simulink model "NBMS_App_Harness1"  (R2026b)
settings: Solver=FixedStepDiscrete  StopTime=25  FixedStep=0.1
undefined symbols (not defined in the file): Active_DisChrg_E, BMS_BattSoCDerate_E, BMS_BattTempDerate_E, BMS_DCDCMosfet_STS_E, BMS_HVMosfet_STS_E, BMS_MODE_E, BMS_NM_Msg_E, BMS_PMosfet_STS_E, Charger_Mode_E, Charger_Mode_Req_E, CV_Mode_Timer_E, OBC_E, VDU_MACHINE_STS_E
(part 4 of 4)

== stateflow chart NBMS_App_Harness1/Test Assessment ==
  state ChargeWhenIgOn
    state step_1
      if t < 0.2
      Expected_BMSMODE = BMS_MODE_E.BMS_SLEEP;
      elseif t >= 0.2 && t < 0.4
      Expected_BMSMODE = BMS_MODE_E.BMS_STANDBY;
      else
      Expected_BMSMODE = BMS_MODE_E.BMS_CHARGE;
      end
      if t < 1.1
      Expected_PrechgMosfet = BMS_PMosfet_STS_E.PDISCONNECTED;
      elseif t >= 1.1 && t < 2.7
      Expected_PrechgMosfet = BMS_PMosfet_STS_E.PCONNECTED;
      else
      Expected_PrechgMosfet = BMS_PMosfet_STS_E.PDISCONNECTED;
      end
      if t < 1.7
      Expected_HVMosfet = BMS_HVMosfet_STS_E.HV_DISCONNECTED;
      elseif t >= 1.7 && t < 2.7
      Expected_HVMosfet = BMS_HVMosfet_STS_E.HV_CONNECT_PENDING;
      else
      Expected_HVMosfet = BMS_HVMosfet_STS_E.HV_CONNECTED;
      end
      if t < 2.2
      Expected_DCDCMosfet = BMS_DCDCMosfet_STS_E.DCDC_DISCONNECTED;
      else
      Expected_DCDCMosfet = BMS_DCDCMosfet_STS_E.DCDC_CONNECTED;
      end
      Expected_ASC_Prep_Flag = false;
      Expected_Chrgr_Prep_Flag = false;
      Expected_PrechgVoltFlt = false;
      verify(AppOut_BMSMODE == Expected_BMSMODE);
      verify(AppOut_PrechgMosfet == Expected_PrechgMosfet);
      verify(AppOut_HVMosfet == Expected_HVMosfet);
      verify(AppOut_DCDCMosfet == Expected_DCDCMosfet);
      verify(AppOut_ASC_Prep_Flag == Expected_ASC_Prep_Flag);
      verify(AppOut_Chrgr_Prep_Flag == Expected_Chrgr_Prep_Flag);
      verify(AppOut_PrechgVoltFlt == Expected_PrechgVoltFlt);
    (default) -> ChargeWhenIgOn.step_1
  state DischgWhenIgOn
    state step_1
      if t < 0.2
      Expected_BMSMODE  = BMS_MODE_E.BMS_SLEEP;
      elseif t >= 0.2 && t < 0.4
      Expected_BMSMODE  = BMS_MODE_E.BMS_STANDBY;
      else
      Expected_BMSMODE  = BMS_MODE_E.BMS_DISCHARGE;
      end
      if t < 1.1
      Expected_PrechgMosfet = BMS_PMosfet_STS_E.PDISCONNECTED;
      elseif t >= 1.1 && t < 2.8
      Expected_PrechgMosfet = BMS_PMosfet_STS_E.PCONNECTED;
      else
      Expected_PrechgMosfet = BMS_PMosfet_STS_E.PDISCONNECTED;
      end
      if t < 1.8
      Expected_HVMosfet = BMS_HVMosfet_STS_E.HV_DISCONNECTED;
      elseif t >= 1.8 && t < 2.8
      Expected_HVMosfet = BMS_HVMosfet_STS_E.HV_CONNECT_PENDING;
      else
      Expected_HVMosfet = BMS_HVMosfet_STS_E.HV_CONNECTED;
      end
      if t < 2.3
      Expected_DCDCMosfet = BMS_DCDCMosfet_STS_E.DCDC_DISCONNECTED;
      else
      Expected_DCDCMosfet = BMS_DCDCMosfet_STS_E.DCDC_CONNECTED;
      end
      Expected_ASC_Prep_Flag = false;
      Expected_Chrgr_Prep_Flag = false;
      Expected_PrechgVoltFlt = false;
      verify(AppOut_BMSMODE == Expected_BMSMODE );
      verify(AppOut_PrechgMosfet == Expected_PrechgMosfet);
      verify(AppOut_HVMosfet == Expected_HVMosfet);
      verify(AppOut_DCDCMosfet == Expected_DCDCMosfet);
      verify(AppOut_ASC_Prep_Flag == Expected_ASC_Prep_Flag);
      verify(AppOut_Chrgr_Prep_Flag == Expected_Chrgr_Prep_Flag);
      verify(AppOut_PrechgVoltFlt == Expected_PrechgVoltFlt);
    (default) -> DischgWhenIgOn.step_1
  state ChargeWhenIgOff
    state step_1
      if t < 0.2
      Expected_BMSMODE  = BMS_MODE_E.BMS_SLEEP;
      elseif t >= 0.2 && t < 0.3
      Expected_BMSMODE  = BMS_MODE_E.BMS_STANDBY;
      else
      Expected_BMSMODE  = BMS_MODE_E.BMS_CHARGE;
      end
      if t < 0.9
      Expected_PrechgMosfet = BMS_PMosfet_STS_E.PDISCONNECTED;
      elseif t >= 0.9 && t < 2.4
      Expected_PrechgMosfet = BMS_PMosfet_STS_E.PCONNECTED;
      else
      Expected_PrechgMosfet = BMS_PMosfet_STS_E.PDISCONNECTED;
      end
      if t < 1.9
      Expected_HVMosfet = BMS_HVMosfet_STS_E.HV_DISCONNECTED;
      elseif t >= 1.9 && t < 2.4
      Expected_HVMosfet = BMS_HVMosfet_STS_E.HV_CONNECT_PENDING;
      else
      Expected_HVMosfet = BMS_HVMosfet_STS_E.HV_CONNECTED;
      end
      Expected_DCDCMosfet = BMS_DCDCMosfet_STS_E.DCDC_DISCONNECTED;
      Expected_ASC_Prep_Flag = false;
      Expected_Chrgr_Prep_Flag = false;
      Expected_PrechgVoltFlt = false;
      verify(AppOut_BMSMODE == Expected_BMSMODE );
      verify(AppOut_PrechgMosfet == Expected_PrechgMosfet);
      verify(AppOut_HVMosfet == Expected_HVMosfet);
      verify(AppOut_DCDCMosfet == Expected_DCDCMosfet);
      verify(AppOut_ASC_Prep_Flag == Expected_ASC_Prep_Flag);
      verify(AppOut_Chrgr_Prep_Flag == Expected_Chrgr_Prep_Flag);
      verify(AppOut_PrechgVoltFlt == Expected_PrechgVoltFlt);
    (default) -> ChargeWhenIgOff.step_1
  state ChgToDischgIgOn
    state step_1
      if t < 0.2
      Expected_BMSMODE  = BMS_MODE_E.BMS_SLEEP;
      elseif t >= 0.2 && t < 0.4
      Expected_BMSMODE  = BMS_MODE_E.BMS_STANDBY;
      elseif t >= 0.4 && t < 4.1
      Expected_BMSMODE  = BMS_MODE_E.BMS_CHARGE;
      elseif t >= 4.1 && t < 4.3
      Expected_BMSMODE  = BMS_MODE_E.BMS_STANDBY;
      else
      Expected_BMSMODE  = BMS_MODE_E.BMS_DISCHARGE;
      end
      if t < 1.1
      Expected_PrechgMosfet = BMS_PMosfet_STS_E.PDISCONNECTED;
      elseif t >= 1.1 && t < 2.8
      Expected_PrechgMosfet = BMS_PMosfet_STS_E.PCONNECTED;
      else
      Expected_PrechgMosfet = BMS_PMosfet_STS_E.PDISCONNECTED;
      end
      if t < 1.8
      Expected_HVMosfet = BMS_HVMosfet_STS_E.HV_DISCONNECTED;
      elseif t >= 1.8 && t < 2.8
      Expected_HVMosfet = BMS_HVMosfet_STS_E.HV_CONNECT_PENDING;
      else
      Expected_HVMosfet = BMS_HVMosfet_STS_E.HV_CONNECTED;
      end
      if t < 2.3
      Expected_DCDCMosfet = BMS_DCDCMosfet_STS_E.DCDC_DISCONNECTED;
      else
      Expected_DCDCMosfet = BMS_DCDCMosfet_STS_E.DCDC_CONNECTED;
      end
      Expected_ASC_Prep_Flag = false;
      Expected_Chrgr_Prep_Flag = false;
      Expected_PrechgVoltFlt = false;
      verify(AppOut_BMSMODE == Expected_BMSMODE );
      verify(AppOut_PrechgMosfet == Expected_PrechgMosfet);
      verify(AppOut_HVMosfet == Expected_HVMosfet);
      verify(AppOut_DCDCMosfet == Expected_DCDCMosfet);
      verify(AppOut_ASC_Prep_Flag == Expected_ASC_Prep_Flag);
      verify(AppOut_Chrgr_Prep_Flag == Expected_Chrgr_Prep_Flag);
      verify(AppOut_PrechgVoltFlt == Expected_PrechgVoltFlt);
    (default) -> ChgToDischgIgOn.step_1
  state SleepToStandby
    state step_1
      if t < 0.2
      Expected_BMSMODE  = BMS_MODE_E.BMS_SLEEP;
      else
      Expected_BMSMODE  = BMS_MODE_E.BMS_STANDBY;
      end
      Expected_PrechgMosfet = BMS_PMosfet_STS_E.PDISCONNECTED;
      Expected_HVMosfet = BMS_HVMosfet_STS_E.HV_DISCONNECTED;
      Expected_DCDCMosfet = BMS_DCDCMosfet_STS_E.DCDC_DISCONNECTED;
      Expected_ASC_Prep_Flag = false;
      Expected_Chrgr_Prep_Flag = false;
      Expected_PrechgVoltFlt = false;
      verify(AppOut_BMSMODE == Expected_BMSMODE );
      verify(AppOut_PrechgMosfet == Expected_PrechgMosfet);
      verify(AppOut_HVMosfet == Expected_HVMosfet);
      verify(AppOut_DCDCMosfet == Expected_DCDCMosfet);
      verify(AppOut_ASC_Prep_Flag == Expected_ASC_Prep_Flag);
      verify(AppOut_Chrgr_Prep_Flag == Expected_Chrgr_Prep_Flag);
      verify(AppOut_PrechgVoltFlt == Expected_PrechgVoltFlt);
    (default) -> SleepToStandby.step_1
  state DischgToStandby
    state step_1
      if t < 0.2
      Expected_BMSMODE  = BMS_MODE_E.BMS_SLEEP;
      elseif t >= 0.2 && t < 0.4
      Expected_BMSMODE  = BMS_MODE_E.BMS_STANDBY;
      elseif t >= 0.4 && t < 3
      Expected_BMSMODE  = BMS_MODE_E.BMS_DISCHARGE;
      elseif t >= 3 && t < 13
      Expected_BMSMODE  = BMS_MODE_E.BMS_STANDBY;
      else
      Expected_BMSMODE  = BMS_MODE_E.BMS_SLEEP;
      end
      if t < 0.8
      Expected_PrechgMosfet = BMS_PMosfet_STS_E.PDISCONNECTED;
      elseif t >= 0.8 && t < 1.9
      Expected_PrechgMosfet = BMS_PMosfet_STS_E.PCONNECTED;
      else
      Expected_PrechgMosfet = BMS_PMosfet_STS_E.PDISCONNECTED;
      end
      if t < 1.3
      Expected_HVMosfet = BMS_HVMosfet_STS_E.HV_DISCONNECTED;
      elseif t >= 1.3 && t < 1.9
      Expected_HVMosfet = BMS_HVMosfet_STS_E.HV_CONNECT_PENDING;
      elseif t >= 1.9 && t < 3.5
      Expected_HVMosfet = BMS_HVMosfet_STS_E.HV_CONNECTED;
      else
      Expected_HVMosfet = BMS_HVMosfet_STS_E.HV_DISCONNECTED;
      end
      if t < 1.6
      Expected_DCDCMosfet = BMS_DCDCMosfet_STS_E.DCDC_DISCONNECTED;
      elseif t >= 1.6 && t < 13
      Expected_DCDCMosfet = BMS_DCDCMosfet_STS_E.DCDC_CONNECTED;
      else
      Expected_DCDCMosfet = BMS_DCDCMosfet_STS_E.DCDC_DISCONNECTED;
      end
      Expected_ASC_Prep_Flag = false;
      Expected_Chrgr_Prep_Flag = false;
      Expected_PrechgVoltFlt = false;
      verify(AppOut_BMSMODE == Expected_BMSMODE );
      verify(AppOut_PrechgMosfet == Expected_PrechgMosfet);
      verify(AppOut_HVMosfet == Expected_HVMosfet);
      verify(AppOut_DCDCMosfet == Expected_DCDCMosfet);
      verify(AppOut_ASC_Prep_Flag == Expected_ASC_Prep_Flag);
      verify(AppOut_Chrgr_Prep_Flag == Expected_Chrgr_Prep_Flag);
      verify(AppOut_PrechgVoltFlt == Expected_PrechgVoltFlt);
    (default) -> DischgToStandby.step_1
  state StandbyToDischgIgOn
    state step_1
      if t < 0.2
      Expected_BMSMODE  = BMS_MODE_E.BMS_SLEEP;
      elseif t >= 0.2 && t < 0.4
      Expected_BMSMODE  = BMS_MODE_E.BMS_STANDBY;
      elseif t >= 0.4 && t < 3
      Expected_BMSMODE  = BMS_MODE_E.BMS_CHARGE;
      elseif t >= 3 && t < 4.8
      Expected_BMSMODE  = BMS_MODE_E.BMS_STANDBY;
      else
      Expected_BMSMODE  = BMS_MODE_E.BMS_DISCHARGE;
      end
      if t < 0.8
      Expected_PrechgMosfet = BMS_PMosfet_STS_E.PDISCONNECTED;
      elseif t >= 0.8 && t < 1.9
      Expected_PrechgMosfet = BMS_PMosfet_STS_E.PCONNECTED;
      elseif t >= 1.9 && t < 5.2
      Expected_PrechgMosfet = BMS_PMosfet_STS_E.PDISCONNECTED;
      elseif t >= 5.2 && t < 6.2
      Expected_PrechgMosfet = BMS_PMosfet_STS_E.PCONNECTED;
      else
      Expected_PrechgMosfet = BMS_PMosfet_STS_E.PDISCONNECTED;
      end
      if t < 1.3
      Expected_HVMosfet = BMS_HVMosfet_STS_E.HV_DISCONNECTED;
      elseif t >= 1.3 && t < 1.9
      Expected_HVMosfet = BMS_HVMosfet_STS_E.HV_CONNECT_PENDING;
      elseif t >= 1.9 && t < 4.5
      Expected_HVMosfet = BMS_HVMosfet_STS_E.HV_CONNECTED;
      elseif t >= 4.5 && t < 5.7
      Expected_HVMosfet = BMS_HVMosfet_STS_E.HV_DISCONNECTED;
      elseif t >= 5.7 && t < 6.2
      Expected_HVMosfet = BMS_HVMosfet_STS_E.HV_CONNECT_PENDING;
      else
      Expected_HVMosfet = BMS_HVMosfet_STS_E.HV_CONNECTED;
      end
      if t < 1.6
      Expected_DCDCMosfet = BMS_DCDCMosfet_STS_E.DCDC_DISCONNECTED;
      else
      Expected_DCDCMosfet = BMS_DCDCMosfet_STS_E.DCDC_CONNECTED;
      end
      Expected_ASC_Prep_Flag = false;
      Expected_Chrgr_Prep_Flag = false;
      Expected_PrechgVoltFlt = false;
      verify(AppOut_BMSMODE == Expected_BMSMODE );
      verify(AppOut_PrechgMosfet == Expected_PrechgMosfet);
      verify(AppOut_HVMosfet == Expected_HVMosfet);
      verify(AppOut_DCDCMosfet == Expected_DCDCMosfet);
      verify(AppOut_ASC_Prep_Flag == Expected_ASC_Prep_Flag);
      verify(AppOut_Chrgr_Prep_Flag == Expected_Chrgr_Prep_Flag);
      verify(AppOut_PrechgVoltFlt == Expected_PrechgVoltFlt);
    (default) -> StandbyToDischgIgOn.step_1
  state IgOffToOnInCharge
    state step_1
      if t < 0.2
      Expected_BMSMODE  = BMS_MODE_E.BMS_SLEEP;
      elseif t >= 0.2 && t < 0.3
      Expected_BMSMODE  = BMS_MODE_E.BMS_STANDBY;
      else
      Expected_BMSMODE  = BMS_MODE_E.BMS_CHARGE;
      end
      if t < 0.6
      Expected_PrechgMosfet = BMS_PMosfet_STS_E.PDISCONNECTED;
      elseif t >= 0.6 && t < 1.6
      Expected_PrechgMosfet = BMS_PMosfet_STS_E.PCONNECTED;
      else
      Expected_PrechgMosfet = BMS_PMosfet_STS_E.PDISCONNECTED;
      end
      if t < 1.1
      Expected_HVMosfet = BMS_HVMosfet_STS_E.HV_DISCONNECTED;
      elseif t >= 1.1 && t < 1.6
      Expected_HVMosfet = BMS_HVMosfet_STS_E.HV_CONNECT_PENDING;
      else
      Expected_HVMosfet = BMS_HVMosfet_STS_E.HV_CONNECTED;
      end
      if t < 2.7
      Expected_DCDCMosfet = BMS_DCDCMosfet_STS_E.DCDC_DISCONNECTED;
      else
      Expected_DCDCMosfet = BMS_DCDCMosfet_STS_E.DCDC_CONNECTED;
      end
      Expected_ASC_Prep_Flag = false;
      Expected_Chrgr_Prep_Flag = false;
      Expected_PrechgVoltFlt = false;
      verify(AppOut_BMSMODE == Expected_BMSMODE );
      verify(AppOut_PrechgMosfet == Expected_PrechgMosfet);
      verify(AppOut_HVMosfet == Expected_HVMosfet);
      verify(AppOut_DCDCMosfet == Expected_DCDCMosfet);
      verify(AppOut_ASC_Prep_Flag == Expected_ASC_Prep_Flag);
      verify(AppOut_Chrgr_Prep_Flag == Expected_Chrgr_Prep_Flag);
      verify(AppOut_PrechgVoltFlt == Expected_PrechgVoltFlt);
    (default) -> IgOffToOnInCharge.step_1
  state IgOnToOffInCharge
    state step_1
      if t < 0.2
      Expected_BMSMODE  = BMS_MODE_E.BMS_SLEEP;
      elseif t >= 0.2 && t < 0.4
      Expected_BMSMODE  = BMS_MODE_E.BMS_STANDBY;
      else
      Expected_BMSMODE  = BMS_MODE_E.BMS_CHARGE;
      end
      if t < 0.8
      Expected_PrechgMosfet = BMS_PMosfet_STS_E.PDISCONNECTED;
      elseif t >= 0.8 && t < 1.9
      Expected_PrechgMosfet = BMS_PMosfet_STS_E.PCONNECTED;
      else
      Expected_PrechgMosfet = BMS_PMosfet_STS_E.PDISCONNECTED;
      end
      if t < 1.3
      Expected_HVMosfet = BMS_HVMosfet_STS_E.HV_DISCONNECTED;
      elseif t >= 1.3 && t < 1.9
      Expected_HVMosfet = BMS_HVMosfet_STS_E.HV_CONNECT_PENDING;
      else
      Expected_HVMosfet = BMS_HVMosfet_STS_E.HV_CONNECTED;
      end
      if t < 1.6
      Expected_DCDCMosfet = BMS_DCDCMosfet_STS_E.DCDC_DISCONNECTED;
      elseif t >= 1.6 && t < 3.3
      Expected_DCDCMosfet = BMS_DCDCMosfet_STS_E.DCDC_CONNECTED;
      else
      Expected_DCDCMosfet = BMS_DCDCMosfet_STS_E.DCDC_DISCONNECTED;
      end
      Expected_ASC_Prep_Flag = false;
      Expected_Chrgr_Prep_Flag = false;
      Expected_PrechgVoltFlt = false;
      verify(AppOut_BMSMODE == Expected_BMSMODE );
      verify(AppOut_PrechgMosfet == Expected_PrechgMosfet);
      verify(AppOut_HVMosfet == Expected_HVMosfet);
      verify(AppOut_DCDCMosfet == Expected_DCDCMosfet);
      verify(AppOut_ASC_Prep_Flag == Expected_ASC_Prep_Flag);
      verify(AppOut_Chrgr_Prep_Flag == Expected_Chrgr_Prep_Flag);
      verify(AppOut_PrechgVoltFlt == Expected_PrechgVoltFlt);
    (default) -> IgOnToOffInCharge.step_1
  state VehPoweredOff
    state step_1
      if t < 0.2
      Expected_BMSMODE  = BMS_MODE_E.BMS_SLEEP;
      elseif t >= 0.2 && t < 0.4
      Expected_BMSMODE  = BMS_MODE_E.BMS_STANDBY;
      elseif t >= 0.4 && t < 3
      Expected_BMSMODE  = BMS_MODE_E.BMS_DISCHARGE;
      elseif t >= 3 && t < 13
      Expected_BMSMODE  = BMS_MODE_E.BMS_STANDBY;
      else
      Expected_BMSMODE  = BMS_MODE_E.BMS_SLEEP;
      end
      if t < 0.8
      Expected_PrechgMosfet = BMS_PMosfet_STS_E.PDISCONNECTED;
      elseif t >= 0.8 && t < 1.9
      Expected_PrechgMosfet = BMS_PMosfet_STS_E.PCONNECTED;
      else
      Expected_PrechgMosfet = BMS_PMosfet_STS_E.PDISCONNECTED;
      end
      if t < 1.3
      Expected_HVMosfet = BMS_HVMosfet_STS_E.HV_DISCONNECTED;
      elseif t >= 1.3 && t < 1.9
      Expected_HVMosfet = BMS_HVMosfet_STS_E.HV_CONNECT_PENDING;
      elseif t >= 1.9 && t < 3.5
      Expected_HVMosfet = BMS_HVMosfet_STS_E.HV_CONNECTED;
      else
      Expected_HVMosfet = BMS_HVMosfet_STS_E.HV_DISCONNECTED;
      end
      if t < 1.6
      Expected_DCDCMosfet = BMS_DCDCMosfet_STS_E.DCDC_DISCONNECTED;
      elseif t >= 1.6 && t < 3.6
      Expected_DCDCMosfet = BMS_DCDCMosfet_STS_E.DCDC_CONNECTED;
      else
      Expected_DCDCMosfet = BMS_DCDCMosfet_STS_E.DCDC_DISCONNECTED;
      end
      Expected_ASC_Prep_Flag = false;
      Expected_Chrgr_Prep_Flag = false;
      Expected_PrechgVoltFlt = false;
      verify(AppOut_BMSMODE == Expected_BMSMODE );
      verify(AppOut_PrechgMosfet == Expected_PrechgMosfet);
      verify(AppOut_HVMosfet == Expected_HVMosfet);
      verify(AppOut_DCDCMosfet == Expected_DCDCMosfet);
      verify(AppOut_ASC_Prep_Flag == Expected_ASC_Prep_Flag);
      verify(AppOut_Chrgr_Prep_Flag == Expected_Chrgr_Prep_Flag);
      verify(AppOut_PrechgVoltFlt == Expected_PrechgVoltFlt);
    (default) -> VehPoweredOff.step_1
  state G4T1DischgFlt
    state step_1
      if t < 0.2
      Expected_BMSMODE  = BMS_MODE_E.BMS_SLEEP;
      elseif t >= 0.2 && t < 0.4
      Expected_BMSMODE  = BMS_MODE_E.BMS_STANDBY;
      elseif t >= 0.4 && t < 3
      Expected_BMSMODE  = BMS_MODE_E.BMS_DISCHARGE;
      else
      Expected_BMSMODE  = BMS_MODE_E.BMS_FAULT;
      end
      if t < 0.8
      Expected_PrechgMosfet = BMS_PMosfet_STS_E.PDISCONNECTED;
      elseif t >= 0.8 && t < 1.9
      Expected_PrechgMosfet = BMS_PMosfet_STS_E.PCONNECTED;
      else
      Expected_PrechgMosfet = BMS_PMosfet_STS_E.PDISCONNECTED;
      end
      if t < 1.3
      Expected_HVMosfet = BMS_HVMosfet_STS_E.HV_DISCONNECTED;
      elseif t >= 1.3 && t < 1.9
      Expected_HVMosfet = BMS_HVMosfet_STS_E.HV_CONNECT_PENDING;
      elseif t >= 1.9 && t < 8.1
      Expected_HVMosfet = BMS_HVMosfet_STS_E.HV_CONNECTED;
      else
      Expected_HVMosfet = BMS_HVMosfet_STS_E.HV_DISCONNECTED;
      end
      if t < 1.6
      Expected_DCDCMosfet = BMS_DCDCMosfet_STS_E.DCDC_DISCONNECTED;
      else
      Expected_DCDCMosfet = BMS_DCDCMosfet_STS_E.DCDC_CONNECTED;
      end
      if t < 3
      Expected_ASC_Prep_Flag = false;
      elseif t >= 3 && t < 8.1
      Expected_ASC_Prep_Flag = true;
      else
      Expected_ASC_Prep_Flag = false;
      end
      Expected_Chrgr_Prep_Flag = false;
      Expected_PrechgVoltFlt = false;
      verify(AppOut_BMSMODE == Expected_BMSMODE );
      verify(AppOut_PrechgMosfet == Expected_PrechgMosfet);
      verify(AppOut_HVMosfet == Expected_HVMosfet);
      verify(AppOut_DCDCMosfet == Expected_DCDCMosfet);
      verify(AppOut_ASC_Prep_Flag == Expected_ASC_Prep_Flag);
      verify(AppOut_Chrgr_Prep_Flag == Expected_Chrgr_Prep_Flag);
      verify(AppOut_PrechgVoltFlt == Expected_PrechgVoltFlt);
    (default) -> G4T1DischgFlt.step_1
  state G4T2DischgFlt
    state step_1
      if t < 0.2
      Expected_BMSMODE  = BMS_MODE_E.BMS_SLEEP;
      elseif t >= 0.2 && t < 0.4
      Expected_BMSMODE  = BMS_MODE_E.BMS_STANDBY;
      elseif t >= 0.4 && t < 3
      Expected_BMSMODE  = BMS_MODE_E.BMS_DISCHARGE;
      else
      Expected_BMSMODE  = BMS_MODE_E.BMS_FAULT;
      end
      if t < 0.8
      Expected_PrechgMosfet = BMS_PMosfet_STS_E.PDISCONNECTED;
      elseif t >= 0.8 && t < 1.9
      Expected_PrechgMosfet = BMS_PMosfet_STS_E.PCONNECTED;
      else
      Expected_PrechgMosfet = BMS_PMosfet_STS_E.PDISCONNECTED;
      end
      if t < 1.3
      Expected_HVMosfet = BMS_HVMosfet_STS_E.HV_DISCONNECTED;
      elseif t >= 1.3 && t < 1.9
      Expected_HVMosfet = BMS_HVMosfet_STS_E.HV_CONNECT_PENDING;
      elseif t >= 1.9 && t < 8.1
      Expected_HVMosfet = BMS_HVMosfet_STS_E.HV_CONNECTED;
      else
      Expected_HVMosfet = BMS_HVMosfet_STS_E.HV_DISCONNECTED;
      end
      if t < 1.6
      Expected_DCDCMosfet = BMS_DCDCMosfet_STS_E.DCDC_DISCONNECTED;
      elseif t >= 1.6 && t < 8.1
      Expected_DCDCMosfet = BMS_DCDCMosfet_STS_E.DCDC_CONNECTED;
      else
      Expected_DCDCMosfet = BMS_DCDCMosfet_STS_E.DCDC_DISCONNECTED;
      end
      if t < 3
      Expected_ASC_Prep_Flag = false;
      elseif t >= 3 && t < 8.1
      Expected_ASC_Prep_Flag = true;
      else
      Expected_ASC_Prep_Flag = false;
      end
      Expected_Chrgr_Prep_Flag = false;
      Expected_PrechgVoltFlt = false;
      verify(AppOut_BMSMODE == Expected_BMSMODE );
      verify(AppOut_PrechgMosfet == Expected_PrechgMosfet);
      verify(AppOut_HVMosfet == Expected_HVMosfet);
      verify(AppOut_DCDCMosfet == Expected_DCDCMosfet);
      verify(AppOut_ASC_Prep_Flag == Expected_ASC_Prep_Flag);
      verify(AppOut_Chrgr_Prep_Flag == Expected_Chrgr_Prep_Flag);
      verify(AppOut_PrechgVoltFlt == Expected_PrechgVoltFlt);
    (default) -> G4T2DischgFlt.step_1
  state G4CommonFlt
    state step_1
      if t < 0.2
      Expected_BMSMODE  = BMS_MODE_E.BMS_SLEEP;
      elseif t >= 0.2 && t < 0.4
      Expected_BMSMODE  = BMS_MODE_E.BMS_STANDBY;
      elseif t >= 0.4 && t < 3
      Expected_BMSMODE  = BMS_MODE_E.BMS_DISCHARGE;
      else
      Expected_BMSMODE  = BMS_MODE_E.BMS_FAULT;
      end
      if t < 0.8
      Expected_PrechgMosfet = BMS_PMosfet_STS_E.PDISCONNECTED;
      elseif t >= 0.8 && t < 1.9
      Expected_PrechgMosfet = BMS_PMosfet_STS_E.PCONNECTED;
      else
      Expected_PrechgMosfet = BMS_PMosfet_STS_E.PDISCONNECTED;
      end
      if t < 1.3
      Expected_HVMosfet = BMS_HVMosfet_STS_E.HV_DISCONNECTED;
      elseif t >= 1.3 && t < 1.9
      Expected_HVMosfet = BMS_HVMosfet_STS_E.HV_CONNECT_PENDING;
      elseif t >= 1.9 && t < 8.1
      Expected_HVMosfet = BMS_HVMosfet_STS_E.HV_CONNECTED;
      else
      Expected_HVMosfet = BMS_HVMosfet_STS_E.HV_DISCONNECTED;
      end
      if t < 1.6
      Expected_DCDCMosfet = BMS_DCDCMosfet_STS_E.DCDC_DISCONNECTED;
      else
      Expected_DCDCMosfet = BMS_DCDCMosfet_STS_E.DCDC_CONNECTED;
      end
      if t < 3
      Expected_ASC_Prep_Flag = false;
      elseif t >= 3 && t < 8.1
      Expected_ASC_Prep_Flag = true;
      else
      Expected_ASC_Prep_Flag = false;
      end
      if t < 3
      Expected_Chrgr_Prep_Flag = false;
      elseif t >= 3 && t < 8.1
      Expected_Chrgr_Prep_Flag = true;
      else
      Expected_Chrgr_Prep_Flag = false;
      end
      Expected_PrechgVoltFlt = false;
      verify(AppOut_BMSMODE == Expected_BMSMODE );
      verify(AppOut_PrechgMosfet == Expected_PrechgMosfet);
      verify(AppOut_HVMosfet == Expected_HVMosfet);
      verify(AppOut_DCDCMosfet == Expected_DCDCMosfet);
      verify(AppOut_ASC_Prep_Flag == Expected_ASC_Prep_Flag);
      verify(AppOut_Chrgr_Prep_Flag == Expected_Chrgr_Prep_Flag);
      verify(AppOut_PrechgVoltFlt == Expected_PrechgVoltFlt);
    (default) -> G4CommonFlt.step_1
  state G4ChargeFlt
    state step_1
      if t < 0.2
      Expected_BMSMODE  = BMS_MODE_E.BMS_SLEEP;
      elseif t >= 0.2 && t < 0.4
      Expected_BMSMODE  = BMS_MODE_E.BMS_STANDBY;
      elseif t >= 0.4 && t < 3
      Expected_BMSMODE  = BMS_MODE_E.BMS_CHARGE;
      else
      Expected_BMSMODE  = BMS_MODE_E.BMS_FAULT;
      end
      if t < 0.8
      Expected_PrechgMosfet = BMS_PMosfet_STS_E.PDISCONNECTED;
      elseif t >= 0.8 && t < 1.9
      Expected_PrechgMosfet = BMS_PMosfet_STS_E.PCONNECTED;
      else
      Expected_PrechgMosfet = BMS_PMosfet_STS_E.PDISCONNECTED;
      end
      if t < 1.3
      Expected_HVMosfet = BMS_HVMosfet_STS_E.HV_DISCONNECTED;
      elseif t >= 1.3 && t < 1.9
      Expected_HVMosfet = BMS_HVMosfet_STS_E.HV_CONNECT_PENDING;
      elseif t >= 1.9 && t < 8.1
      Expected_HVMosfet = BMS_HVMosfet_STS_E.HV_CONNECTED;
      else
      Expected_HVMosfet = BMS_HVMosfet_STS_E.HV_DISCONNECTED;
      end
      if t < 1.6
      Expected_DCDCMosfet = BMS_DCDCMosfet_STS_E.DCDC_DISCONNECTED;
      else
      Expected_DCDCMosfet = BMS_DCDCMosfet_STS_E.DCDC_CONNECTED;
      end
      Expected_ASC_Prep_Flag = false;
      if t < 3
      Expected_Chrgr_Prep_Flag = false;
      elseif t >= 3 && t < 8.1
      Expected_Chrgr_Prep_Flag = true;
      else
      Expected_Chrgr_Prep_Flag = false;
      end
      Expected_PrechgVoltFlt = false;
      verify(AppOut_BMSMODE == Expected_BMSMODE );
      verify(AppOut_PrechgMosfet == Expected_PrechgMosfet);
      verify(AppOut_HVMosfet == Expected_HVMosfet);
      verify(AppOut_DCDCMosfet == Expected_DCDCMosfet);
      verify(AppOut_ASC_Prep_Flag == Expected_ASC_Prep_Flag);
      verify(AppOut_Chrgr_Prep_Flag == Expected_Chrgr_Prep_Flag);
      verify(AppOut_PrechgVoltFlt == Expected_PrechgVoltFlt);
    (default) -> G4ChargeFlt.step_1
  state DischgToChgIgOn
    state step_1
      if t < 0.2
      Expected_BMSMODE  = BMS_MODE_E.BMS_SLEEP;
      elseif t >= 0.2 && t < 0.4
      Expected_BMSMODE  = BMS_MODE_E.BMS_STANDBY;
      elseif t >= 0.4 && t < 3
      Expected_BMSMODE  = BMS_MODE_E.BMS_DISCHARGE;
      elseif t >= 3 && t < 3.1
      Expected_BMSMODE  = BMS_MODE_E.BMS_STANDBY;
      else
      Expected_BMSMODE  = BMS_MODE_E.BMS_CHARGE;
      end
      if t < 0.8
      Expected_PrechgMosfet = BMS_PMosfet_STS_E.PDISCONNECTED;
      elseif t >= 0.8 && t < 1.9
      Expected_PrechgMosfet = BMS_PMosfet_STS_E.PCONNECTED;
      else
      Expected_PrechgMosfet = BMS_PMosfet_STS_E.PDISCONNECTED;
      end
      if t < 1.3
      Expected_HVMosfet = BMS_HVMosfet_STS_E.HV_DISCONNECTED;
      elseif t >= 1.3 && t < 1.9
      Expected_HVMosfet = BMS_HVMosfet_STS_E.HV_CONNECT_PENDING;
      else
      Expected_HVMosfet = BMS_HVMosfet_STS_E.HV_CONNECTED;
      end
      if t < 1.6
      Expected_DCDCMosfet = BMS_DCDCMosfet_STS_E.DCDC_DISCONNECTED;
      else
      Expected_DCDCMosfet = BMS_DCDCMosfet_STS_E.DCDC_CONNECTED;
      end
      Expected_ASC_Prep_Flag = false;
      Expected_Chrgr_Prep_Flag = false;
      Expected_PrechgVoltFlt = false;
      verify(AppOut_BMSMODE == Expected_BMSMODE );
      verify(AppOut_PrechgMosfet == Expected_PrechgMosfet);
      verify(AppOut_HVMosfet == Expected_HVMosfet);
      verify(AppOut_DCDCMosfet == Expected_DCDCMosfet);
      verify(AppOut_ASC_Prep_Flag == Expected_ASC_Prep_Flag);
      verify(AppOut_Chrgr_Prep_Flag == Expected_Chrgr_Prep_Flag);
      verify(AppOut_PrechgVoltFlt == Expected_PrechgVoltFlt);
    (default) -> DischgToChgIgOn.step_1
  state FaultToSleep
    state step_1
      if t < 0.2
      Expected_BMSMODE  = BMS_MODE_E.BMS_SLEEP;
      elseif t >= 0.2 && t < 0.4
      Expected_BMSMODE  = BMS_MODE_E.BMS_STANDBY;
      elseif t >= 0.4 && t < 3
      Expected_BMSMODE  = BMS_MODE_E.BMS_DISCHARGE;
      elseif t >= 3 && t < 13
      Expected_BMSMODE  = BMS_MODE_E.BMS_FAULT;
      else
      Expected_BMSMODE  = BMS_MODE_E.BMS_SLEEP;
      end
      if t < 0.8
      Expected_PrechgMosfet = BMS_PMosfet_STS_E.PDISCONNECTED;
      elseif t >= 0.8 && t < 1.9
      Expected_PrechgMosfet = BMS_PMosfet_STS_E.PCONNECTED;
      else
      Expected_PrechgMosfet = BMS_PMosfet_STS_E.PDISCONNECTED;
      end
      if t < 1.3
      Expected_HVMosfet = BMS_HVMosfet_STS_E.HV_DISCONNECTED;
      elseif t >= 1.3 && t < 1.9
      Expected_HVMosfet = BMS_HVMosfet_STS_E.HV_CONNECT_PENDING;
      elseif t >= 1.9 && t < 8.1
      Expected_HVMosfet = BMS_HVMosfet_STS_E.HV_CONNECTED;
      else
      Expected_HVMosfet = BMS_HVMosfet_STS_E.HV_DISCONNECTED;
      end
      if t < 1.6
      Expected_DCDCMosfet = BMS_DCDCMosfet_STS_E.DCDC_DISCONNECTED;
      elseif t >= 1.6 && t < 13
      Expected_DCDCMosfet = BMS_DCDCMosfet_STS_E.DCDC_CONNECTED;
      else
      Expected_DCDCMosfet = BMS_DCDCMosfet_STS_E.DCDC_DISCONNECTED;
      end
      if t < 3
      Expected_ASC_Prep_Flag = false;
      elseif t >= 3 && t < 8.1
      Expected_ASC_Prep_Flag = true;
      else
      Expected_ASC_Prep_Flag = false;
      end
      Expected_Chrgr_Prep_Flag = false;
      Expected_PrechgVoltFlt = false;
      verify(AppOut_BMSMODE == Expected_BMSMODE );
      verify(AppOut_PrechgMosfet == Expected_PrechgMosfet);
      verify(AppOut_HVMosfet == Expected_HVMosfet);
      verify(AppOut_DCDCMosfet == Expected_DCDCMosfet);
      verify(AppOut_ASC_Prep_Flag == Expected_ASC_Prep_Flag);
      verify(AppOut_Chrgr_Prep_Flag == Expected_Chrgr_Prep_Flag);
      verify(AppOut_PrechgVoltFlt == Expected_PrechgVoltFlt);
    (default) -> FaultToSleep.step_1
  state ChgToStandbyIgOn
    state step_1
      if t < 0.2
      Expected_BMSMODE  = BMS_MODE_E.BMS_SLEEP;
      elseif t >= 0.2 && t < 0.4
      Expected_BMSMODE  = BMS_MODE_E.BMS_STANDBY;
      elseif t >= 0.4 && t < 3
      Expected_BMSMODE  = BMS_MODE_E.BMS_CHARGE;
      else
      Expected_BMSMODE  = BMS_MODE_E.BMS_STANDBY;
      end
      if t < 0.8
      Expected_PrechgMosfet = BMS_PMosfet_STS_E.PDISCONNECTED;
      elseif t >= 0.8 && t < 1.9
      Expected_PrechgMosfet = BMS_PMosfet_STS_E.PCONNECTED;
      else
      Expected_PrechgMosfet = BMS_PMosfet_STS_E.PDISCONNECTED;
      end
      if t < 1.3
      Expected_HVMosfet = BMS_HVMosfet_STS_E.HV_DISCONNECTED;
      elseif t >= 1.3 && t < 1.9
      Expected_HVMosfet = BMS_HVMosfet_STS_E.HV_CONNECT_PENDING;
      elseif t >= 1.9 && t < 3.5
      Expected_HVMosfet = BMS_HVMosfet_STS_E.HV_CONNECTED;
      else
      Expected_HVMosfet = BMS_HVMosfet_STS_E.HV_DISCONNECTED;
      end
      if t < 1.6
      Expected_DCDCMosfet = BMS_DCDCMosfet_STS_E.DCDC_DISCONNECTED;
      else
      Expected_DCDCMosfet = BMS_DCDCMosfet_STS_E.DCDC_CONNECTED;
      end
      Expected_ASC_Prep_Flag = false;
      Expected_Chrgr_Prep_Flag = false;
      Expected_PrechgVoltFlt = false;
      verify(AppOut_BMSMODE == Expected_BMSMODE );
      verify(AppOut_PrechgMosfet == Expected_PrechgMosfet);
      verify(AppOut_HVMosfet == Expected_HVMosfet);
      verify(AppOut_DCDCMosfet == Expected_DCDCMosfet);
      verify(AppOut_ASC_Prep_Flag == Expected_ASC_Prep_Flag);
      verify(AppOut_Chrgr_Prep_Flag == Expected_Chrgr_Prep_Flag);
      verify(AppOut_PrechgVoltFlt == Expected_PrechgVoltFlt);
    (default) -> ChgToStandbyIgOn.step_1
  state ChgToStandbyIgOff
    state step_1
      if t < 0.2
      Expected_BMSMODE  = BMS_MODE_E.BMS_SLEEP;
      elseif t >= 0.2 && t < 0.3
      Expected_BMSMODE  = BMS_MODE_E.BMS_STANDBY;
      elseif t >= 0.3 && t < 2.7
      Expected_BMSMODE  = BMS_MODE_E.BMS_CHARGE;
      elseif t >= 2.7 && t < 12.7
      Expected_BMSMODE  = BMS_MODE_E.BMS_STANDBY;
      else
      Expected_BMSMODE  = BMS_MODE_E.BMS_SLEEP;
      end
      if t < 0.6
      Expected_PrechgMosfet = BMS_PMosfet_STS_E.PDISCONNECTED;
      elseif t >= 0.6 && t < 1.6
      Expected_PrechgMosfet = BMS_PMosfet_STS_E.PCONNECTED;
      else
      Expected_PrechgMosfet = BMS_PMosfet_STS_E.PDISCONNECTED;
      end
      if t < 1.1
      Expected_HVMosfet = BMS_HVMosfet_STS_E.HV_DISCONNECTED;
      elseif t >= 1.1 && t < 1.6
      Expected_HVMosfet = BMS_HVMosfet_STS_E.HV_CONNECT_PENDING;
      elseif t >= 1.6 && t < 3.2
      Expected_HVMosfet = BMS_HVMosfet_STS_E.HV_CONNECTED;
      else
      Expected_HVMosfet = BMS_HVMosfet_STS_E.HV_DISCONNECTED;
      end
      Expected_DCDCMosfet = BMS_DCDCMosfet_STS_E.DCDC_DISCONNECTED;
      Expected_ASC_Prep_Flag = false;
      Expected_Chrgr_Prep_Flag = false;
      Expected_PrechgVoltFlt = false;
      verify(AppOut_BMSMODE == Expected_BMSMODE );
      verify(AppOut_PrechgMosfet == Expected_PrechgMosfet);
      verify(AppOut_HVMosfet == Expected_HVMosfet);
      verify(AppOut_DCDCMosfet == Expected_DCDCMosfet);
      verify(AppOut_ASC_Prep_Flag == Expected_ASC_Prep_Flag);
      verify(AppOut_Chrgr_Prep_Flag == Expected_Chrgr_Prep_Flag);
      verify(AppOut_PrechgVoltFlt == Expected_PrechgVoltFlt);
    (default) -> ChgToStandbyIgOff.step_1
  state StandbyToChargeIgOn
    state step_1
      if t < 0.2
      Expected_BMSMODE  = BMS_MODE_E.BMS_SLEEP;
      elseif t >= 0.2 && t < 0.4
      Expected_BMSMODE  = BMS_MODE_E.BMS_STANDBY;
      elseif t >= 0.4 && t < 3
      Expected_BMSMODE  = BMS_MODE_E.BMS_DISCHARGE;
      elseif t >= 3 && t < 3.9
      Expected_BMSMODE  = BMS_MODE_E.BMS_STANDBY;
      else
      Expected_BMSMODE  = BMS_MODE_E.BMS_CHARGE;
      end
      if t < 0.8
      Expected_PrechgMosfet = BMS_PMosfet_STS_E.PDISCONNECTED;
      elseif t >= 0.8 && t < 1.9
      Expected_PrechgMosfet = BMS_PMosfet_STS_E.PCONNECTED;
      elseif t >= 1.9 && t < 4.3
      Expected_PrechgMosfet = BMS_PMosfet_STS_E.PDISCONNECTED;
      elseif t >= 4.3 && t < 5.2
      Expected_PrechgMosfet = BMS_PMosfet_STS_E.PCONNECTED;
      else
      Expected_PrechgMosfet = BMS_PMosfet_STS_E.PDISCONNECTED;
      end
      if t < 1.3
      Expected_HVMosfet = BMS_HVMosfet_STS_E.HV_DISCONNECTED;
      elseif t >= 1.3 && t < 1.9
      Expected_HVMosfet = BMS_HVMosfet_STS_E.HV_CONNECT_PENDING;
      elseif t >= 1.9 && t < 3.5
      Expected_HVMosfet = BMS_HVMosfet_STS_E.HV_CONNECTED;
      elseif t >= 3.5 && t < 4.7
      Expected_HVMosfet = BMS_HVMosfet_STS_E.HV_DISCONNECTED;
      elseif t >= 4.7 && t < 5.2
      Expected_HVMosfet = BMS_HVMosfet_STS_E.HV_CONNECT_PENDING;
      else
      Expected_HVMosfet = BMS_HVMosfet_STS_E.HV_CONNECTED;
      end
      if t < 1.6
      Expected_DCDCMosfet = BMS_DCDCMosfet_STS_E.DCDC_DISCONNECTED;
      else
      Expected_DCDCMosfet = BMS_DCDCMosfet_STS_E.DCDC_CONNECTED;
      end
      Expected_ASC_Prep_Flag = false;
      Expected_Chrgr_Prep_Flag = false;
      Expected_PrechgVoltFlt = false;
      verify(AppOut_BMSMODE == Expected_BMSMODE );
      verify(AppOut_PrechgMosfet == Expected_PrechgMosfet);
      verify(AppOut_HVMosfet == Expected_HVMosfet);
      verify(AppOut_DCDCMosfet == Expected_DCDCMosfet);
      verify(AppOut_ASC_Prep_Flag == Expected_ASC_Prep_Flag);
      verify(AppOut_Chrgr_Prep_Flag == Expected_Chrgr_Prep_Flag);
      verify(AppOut_PrechgVoltFlt == Expected_PrechgVoltFlt);
    (default) -> StandbyToChargeIgOn.step_1
  state StandbyToChargeIgOff
    state step_1
      if t < 0.2
      Expected_BMSMODE  = BMS_MODE_E.BMS_SLEEP;
      elseif t >= 0.2 && t < 0.4
      Expected_BMSMODE  = BMS_MODE_E.BMS_STANDBY;
      elseif t >= 0.4 && t < 3
      Expected_BMSMODE  = BMS_MODE_E.BMS_DISCHARGE;
      elseif t >= 3 && t < 3.9
      Expected_BMSMODE  = BMS_MODE_E.BMS_STANDBY;
      else
      Expected_BMSMODE  = BMS_MODE_E.BMS_CHARGE;
      end
      if t < 0.8
      Expected_PrechgMosfet = BMS_PMosfet_STS_E.PDISCONNECTED;
      elseif t >= 0.8 && t < 1.9
      Expected_PrechgMosfet = BMS_PMosfet_STS_E.PCONNECTED;
      elseif t >= 1.9 && t < 4.3
      Expected_PrechgMosfet = BMS_PMosfet_STS_E.PDISCONNECTED;
      elseif t >= 4.3 && t < 5.3
      Expected_PrechgMosfet = BMS_PMosfet_STS_E.PCONNECTED;
      else
      Expected_PrechgMosfet = BMS_PMosfet_STS_E.PDISCONNECTED;
      end
      if t < 1.3
      Expected_HVMosfet = BMS_HVMosfet_STS_E.HV_DISCONNECTED;
      elseif t >= 1.3 && t < 1.9
      Expected_HVMosfet = BMS_HVMosfet_STS_E.HV_CONNECT_PENDING;
      elseif t >= 1.9 && t < 3.5
      Expected_HVMosfet = BMS_HVMosfet_STS_E.HV_CONNECTED;
      elseif t >= 3.5 && t < 4.7
      Expected_HVMosfet = BMS_HVMosfet_STS_E.HV_DISCONNECTED;
      elseif t >= 4.7 && t < 5.3
      Expected_HVMosfet = BMS_HVMosfet_STS_E.HV_CONNECT_PENDING;
      else
      Expected_HVMosfet = BMS_HVMosfet_STS_E.HV_CONNECTED;
      end
      if t < 1.6
      Expected_DCDCMosfet = BMS_DCDCMosfet_STS_E.DCDC_DISCONNECTED;
      elseif t >= 1.6 && t < 5
      Expected_DCDCMosfet = BMS_DCDCMosfet_STS_E.DCDC_CONNECTED;
      else
      Expected_DCDCMosfet = BMS_DCDCMosfet_STS_E.DCDC_DISCONNECTED;
      end
      Expected_ASC_Prep_Flag = false;
      Expected_Chrgr_Prep_Flag = false;
      Expected_PrechgVoltFlt = false;
      verify(AppOut_BMSMODE == Expected_BMSMODE );
      verify(AppOut_PrechgMosfet == Expected_PrechgMosfet);
      verify(AppOut_HVMosfet == Expected_HVMosfet);
      verify(AppOut_DCDCMosfet == Expected_DCDCMosfet);
      verify(AppOut_ASC_Prep_Flag == Expected_ASC_Prep_Flag);
      verify(AppOut_Chrgr_Prep_Flag == Expected_Chrgr_Prep_Flag);
      verify(AppOut_PrechgVoltFlt == Expected_PrechgVoltFlt);
    (default) -> StandbyToChargeIgOff.step_1
  state ChgToFltIgOff
    state step_1
      if t < 0.2
      Expected_BMSMODE  = BMS_MODE_E.BMS_SLEEP;
      elseif t >= 0.2 && t < 0.3
      Expected_BMSMODE  = BMS_MODE_E.BMS_STANDBY;
      elseif t >= 0.3 && t < 2.7
      Expected_BMSMODE  = BMS_MODE_E.BMS_CHARGE;
      elseif t >= 2.7 && t < 12.7
      Expected_BMSMODE  = BMS_MODE_E.BMS_FAULT;
      else
      Expected_BMSMODE  = BMS_MODE_E.BMS_SLEEP;
      end
      if t < 0.6
      Expected_PrechgMosfet = BMS_PMosfet_STS_E.PDISCONNECTED;
      elseif t >= 0.6 && t < 1.6
      Expected_PrechgMosfet = BMS_PMosfet_STS_E.PCONNECTED;
      else
      Expected_PrechgMosfet = BMS_PMosfet_STS_E.PDISCONNECTED;
      end
      if t < 1.1
      Expected_HVMosfet = BMS_HVMosfet_STS_E.HV_DISCONNECTED;
      elseif t >= 1.1 && t < 1.6
      Expected_HVMosfet = BMS_HVMosfet_STS_E.HV_CONNECT_PENDING;
      elseif t >= 1.6 && t < 7.8
      Expected_HVMosfet = BMS_HVMosfet_STS_E.HV_CONNECTED;
      else
      Expected_HVMosfet = BMS_HVMosfet_STS_E.HV_DISCONNECTED;
      end
      Expected_DCDCMosfet = BMS_DCDCMosfet_STS_E.DCDC_DISCONNECTED;
      Expected_ASC_Prep_Flag = false;
      if t < 2.7
      Expected_Chrgr_Prep_Flag = false;
      elseif t >= 2.7 && t < 7.8
      Expected_Chrgr_Prep_Flag = true;
      else
      Expected_Chrgr_Prep_Flag = false;
      end
      Expected_PrechgVoltFlt = false;
      verify(AppOut_BMSMODE == Expected_BMSMODE );
      verify(AppOut_PrechgMosfet == Expected_PrechgMosfet);
      verify(AppOut_HVMosfet == Expected_HVMosfet);
      verify(AppOut_DCDCMosfet == Expected_DCDCMosfet);
      verify(AppOut_ASC_Prep_Flag == Expected_ASC_Prep_Flag);
      verify(AppOut_Chrgr_Prep_Flag == Expected_Chrgr_Prep_Flag);
      verify(AppOut_PrechgVoltFlt == Expected_PrechgVoltFlt);
    (default) -> ChgToFltIgOff.step_1
  state FltToChgIgOff
    state step_1
      if t < 0.2
      Expected_BMSMODE  = BMS_MODE_E.BMS_SLEEP;
      elseif t >= 0.2 && t < 0.4
      Expected_BMSMODE  = BMS_MODE_E.BMS_STANDBY;
      elseif t >= 0.4 && t < 3
      Expected_BMSMODE  = BMS_MODE_E.BMS_DISCHARGE;
      elseif t >= 3 && t < 9.2
      Expected_BMSMODE  = BMS_MODE_E.BMS_FAULT;
      else
      Expected_BMSMODE  = BMS_MODE_E.BMS_CHARGE;
      end
      if t < 0.8
      Expected_PrechgMosfet = BMS_PMosfet_STS_E.PDISCONNECTED;
      elseif t >= 0.8 && t < 1.9
      Expected_PrechgMosfet = BMS_PMosfet_STS_E.PCONNECTED;
      elseif t >= 1.9 && t < 9.6
      Expected_PrechgMosfet = BMS_PMosfet_STS_E.PDISCONNECTED;
      elseif t >= 9.6 && t < 10.6
      Expected_PrechgMosfet = BMS_PMosfet_STS_E.PCONNECTED;
      else
      Expected_PrechgMosfet = BMS_PMosfet_STS_E.PDISCONNECTED;
      end
      if t < 1.3
      Expected_HVMosfet = BMS_HVMosfet_STS_E.HV_DISCONNECTED;
      elseif t >= 1.3 && t < 1.9
      Expected_HVMosfet = BMS_HVMosfet_STS_E.HV_CONNECT_PENDING;
      elseif t >= 1.9 && t < 8.1
      Expected_HVMosfet = BMS_HVMosfet_STS_E.HV_CONNECTED;
      elseif t >= 8.1 && t < 9.9
      Expected_HVMosfet = BMS_HVMosfet_STS_E.HV_DISCONNECTED;
      elseif t >= 9.9 && t < 10.6
      Expected_HVMosfet = BMS_HVMosfet_STS_E.HV_CONNECT_PENDING;
      else
      Expected_HVMosfet = BMS_HVMosfet_STS_E.HV_CONNECTED;
      end
      if t < 1.6
      Expected_DCDCMosfet = BMS_DCDCMosfet_STS_E.DCDC_DISCONNECTED;
      elseif t >= 1.6 && t < 8.1
      Expected_DCDCMosfet = BMS_DCDCMosfet_STS_E.DCDC_CONNECTED;
      else
      Expected_DCDCMosfet = BMS_DCDCMosfet_STS_E.DCDC_DISCONNECTED;
      end
      if t < 3
      Expected_ASC_Prep_Flag = false;
      elseif t >= 3 && t < 8.1
      Expected_ASC_Prep_Flag = true;
      else
      Expected_ASC_Prep_Flag = false;
      end
      Expected_Chrgr_Prep_Flag = false;
      Expected_PrechgVoltFlt = false;
      verify(AppOut_BMSMODE == Expected_BMSMODE );
      verify(AppOut_PrechgMosfet == Expected_PrechgMosfet);
      verify(AppOut_HVMosfet == Expected_HVMosfet);
      verify(AppOut_DCDCMosfet == Expected_DCDCMosfet);
      verify(AppOut_ASC_Prep_Flag == Expected_ASC_Prep_Flag);
      verify(AppOut_Chrgr_Prep_Flag == Expected_Chrgr_Prep_Flag);
      verify(AppOut_PrechgVoltFlt == Expected_PrechgVoltFlt);
    (default) -> FltToChgIgOff.step_1
  state FltToChgIgOn
    state step_1
      if t < 0.2
      Expected_BMSMODE  = BMS_MODE_E.BMS_SLEEP;
      elseif t >= 0.2 && t < 0.4
      Expected_BMSMODE  = BMS_MODE_E.BMS_STANDBY;
      elseif t >= 0.4 && t < 3
      Expected_BMSMODE  = BMS_MODE_E.BMS_DISCHARGE;
      elseif t >= 3 && t < 9.2
      Expected_BMSMODE  = BMS_MODE_E.BMS_FAULT;
      else
      Expected_BMSMODE  = BMS_MODE_E.BMS_CHARGE;
      end
      if t < 0.8
      Expected_PrechgMosfet = BMS_PMosfet_STS_E.PDISCONNECTED;
      elseif t >= 0.8 && t < 1.9
      Expected_PrechgMosfet = BMS_PMosfet_STS_E.PCONNECTED;
      elseif t >= 1.9 && t < 9.6
      Expected_PrechgMosfet = BMS_PMosfet_STS_E.PDISCONNECTED;
      elseif t >= 9.6 && t < 10.5
      Expected_PrechgMosfet = BMS_PMosfet_STS_E.PCONNECTED;
      else
      Expected_PrechgMosfet = BMS_PMosfet_STS_E.PDISCONNECTED;
      end
      if t < 1.3
      Expected_HVMosfet = BMS_HVMosfet_STS_E.HV_DISCONNECTED;
      elseif t >= 1.3 && t < 1.9
      Expected_HVMosfet = BMS_HVMosfet_STS_E.HV_CONNECT_PENDING;
      elseif t >= 1.9 && t < 8.1
      Expected_HVMosfet = BMS_HVMosfet_STS_E.HV_CONNECTED;
      elseif t >= 8.1 && t < 9.9
      Expected_HVMosfet = BMS_HVMosfet_STS_E.HV_DISCONNECTED;
      elseif t >= 9.9 && t < 10.5
      Expected_HVMosfet = BMS_HVMosfet_STS_E.HV_CONNECT_PENDING;
      else
      Expected_HVMosfet = BMS_HVMosfet_STS_E.HV_CONNECTED;
      end
      if t < 1.6
      Expected_DCDCMosfet = BMS_DCDCMosfet_STS_E.DCDC_DISCONNECTED;
      else
      Expected_DCDCMosfet = BMS_DCDCMosfet_STS_E.DCDC_CONNECTED;
      end
      if t < 3
      Expected_ASC_Prep_Flag = false;
      elseif t >= 3 && t < 8.1
      Expected_ASC_Prep_Flag = true;
      else
      Expected_ASC_Prep_Flag = false;
      end
      Expected_Chrgr_Prep_Flag = false;
      Expected_PrechgVoltFlt = false;
      verify(AppOut_BMSMODE == Expected_BMSMODE );
      verify(AppOut_PrechgMosfet == Expected_PrechgMosfet);
      verify(AppOut_HVMosfet == Expected_HVMosfet);
      verify(AppOut_DCDCMosfet == Expected_DCDCMosfet);
      verify(AppOut_ASC_Prep_Flag == Expected_ASC_Prep_Flag);
      verify(AppOut_Chrgr_Prep_Flag == Expected_Chrgr_Prep_Flag);
      verify(AppOut_PrechgVoltFlt == Expected_PrechgVoltFlt);
    (default) -> FltToChgIgOn.step_1
  state PrechgVoltFltWhenIgOn
    state step_1
      if t < 0.2
      Expected_BMSMODE  = BMS_MODE_E.BMS_SLEEP;
      elseif t >= 0.2 && t < 0.3
      Expected_BMSMODE  = BMS_MODE_E.BMS_STANDBY;
      elseif t >= 0.3 && t < 1.2
      Expected_BMSMODE  = BMS_MODE_E.BMS_DISCHARGE;
      else
      Expected_BMSMODE  = BMS_MODE_E.BMS_FAULT;
      end
      if t < 0.6
      Expected_PrechgMosfet = BMS_PMosfet_STS_E.PDISCONNECTED;
      elseif t >= 0.6 && t < 1.0
      Expected_PrechgMosfet = BMS_PMosfet_STS_E.PCONNECTED;
      elseif t >= 1.0&& t < 6.2
      Expected_PrechgMosfet = BMS_PMosfet_STS_E.PMOSFET_FAULT;
      else
      Expected_PrechgMosfet = BMS_PMosfet_STS_E.PDISCONNECTED;
      end
      Expected_HVMosfet = BMS_HVMosfet_STS_E.HV_DISCONNECTED
      Expected_DCDCMosfet = BMS_DCDCMosfet_STS_E.DCDC_DISCONNECTED
      if t < 1.1
      Expected_ASC_Prep_Flag = false;
      elseif t >= 1.1 && t < 6.2
      Expected_ASC_Prep_Flag = true;
      else
      Expected_ASC_Prep_Flag = false;
      end
      if t < 1.1
      Expected_Chrgr_Prep_Flag = false;
      elseif t >= 1.1 && t < 6.2
      Expected_Chrgr_Prep_Flag = true;
      else
      Expected_Chrgr_Prep_Flag = false;
      end
      if t < 1.0
      Expected_PrechgVoltFlt= false;
      elseif t >= 1.0 && t < 6.2
      Expected_PrechgVoltFlt= true;
      else
      Expected_PrechgVoltFlt= false;
      end
      verify(AppOut_BMSMODE == Expected_BMSMODE );
      verify(AppOut_PrechgMosfet == Expected_PrechgMosfet);
      verify(AppOut_HVMosfet == Expected_HVMosfet);
      verify(AppOut_DCDCMosfet == Expected_DCDCMosfet);
      verify(AppOut_ASC_Prep_Flag == Expected_ASC_Prep_Flag);
      verify(AppOut_Chrgr_Prep_Flag == Expected_Chrgr_Prep_Flag);
      verify(AppOut_PrechgVoltFlt == Expected_PrechgVoltFlt);
    (default) -> PrechgVoltFltWhenIgOn.step_1
  state PrechgVoltFltWhenIgOff
    state step_1
      if t < 0.2
      Expected_BMSMODE  = BMS_MODE_E.BMS_SLEEP;
      elseif t >= 0.2 && t < 0.3
      Expected_BMSMODE  = BMS_MODE_E.BMS_STANDBY;
      elseif t >= 0.3 && t < 1.2
      Expected_BMSMODE  = BMS_MODE_E.BMS_CHARGE;
      else
      Expected_BMSMODE  = BMS_MODE_E.BMS_FAULT;
      end
      if t < 0.6
      Expected_PrechgMosfet = BMS_PMosfet_STS_E.PDISCONNECTED;
      elseif t >= 0.6 && t < 1.0
      Expected_PrechgMosfet = BMS_PMosfet_STS_E.PCONNECTED;
      elseif t >= 1.0&& t < 6.2
      Expected_PrechgMosfet = BMS_PMosfet_STS_E.PMOSFET_FAULT;
      else
      Expected_PrechgMosfet = BMS_PMosfet_STS_E.PDISCONNECTED;
      end
      Expected_HVMosfet = BMS_HVMosfet_STS_E.HV_DISCONNECTED
      Expected_DCDCMosfet = BMS_DCDCMosfet_STS_E.DCDC_DISCONNECTED
      if t < 1.1
      Expected_ASC_Prep_Flag = false;
      elseif t >= 1.1 && t < 6.2
      Expected_ASC_Prep_Flag = true;
      else
      Expected_ASC_Prep_Flag = false;
      end
      if t < 1.1
      Expected_Chrgr_Prep_Flag = false;
      elseif t >= 1.1 && t < 6.2
      Expected_Chrgr_Prep_Flag = true;
      else
      Expected_Chrgr_Prep_Flag = false;
      end
      if t < 1.0
      Expected_PrechgVoltFlt= false;
      elseif t >= 1.0 && t < 6.2
      Expected_PrechgVoltFlt= true;
      else
      Expected_PrechgVoltFlt= false;
      end
      verify(AppOut_BMSMODE == Expected_BMSMODE );
      verify(AppOut_PrechgMosfet == Expected_PrechgMosfet);
      verify(AppOut_HVMosfet == Expected_HVMosfet);
      verify(AppOut_DCDCMosfet == Expected_DCDCMosfet);
      verify(AppOut_ASC_Prep_Flag == Expected_ASC_Prep_Flag);
      verify(AppOut_Chrgr_Prep_Flag == Expected_Chrgr_Prep_Flag);
      verify(AppOut_PrechgVoltFlt == Expected_PrechgVoltFlt);
    (default) -> PrechgVoltFltWhenIgOff.step_1
  state ChargeSequenceIgOff
    state step_1
      if t < 0.2
      Expected_BMSMODE  = BMS_MODE_E.BMS_SLEEP;
      elseif t >= 0.2 && t < 0.3
      Expected_BMSMODE  = BMS_MODE_E.BMS_STANDBY;
      else
      Expected_BMSMODE  = BMS_MODE_E.BMS_CHARGE;
      end
      if t < 0.6
      Expected_PrechgMosfet = BMS_PMosfet_STS_E.PDISCONNECTED;
      elseif t >= 0.6 && t < 1.6
      Expected_PrechgMosfet = BMS_PMosfet_STS_E.PCONNECTED;
      else
      Expected_PrechgMosfet = BMS_PMosfet_STS_E.PDISCONNECTED;
      end
      if t < 1.1
      Expected_HVMosfet = BMS_HVMosfet_STS_E.HV_DISCONNECTED;
      elseif t >= 1.1 && t < 1.6
      Expected_HVMosfet = BMS_HVMosfet_STS_E.HV_CONNECT_PENDING;
      else
      Expected_HVMosfet = BMS_HVMosfet_STS_E.HV_CONNECTED;
      end
      if t < 2.7
      Expected_DCDCMosfet = BMS_DCDCMosfet_STS_E.DCDC_DISCONNECTED;
      elseif t >= 2.7 && t < 2.9
      Expected_DCDCMosfet = BMS_DCDCMosfet_STS_E.DCDC_CONNECTED;
      else
      Expected_DCDCMosfet = BMS_DCDCMosfet_STS_E.DCDC_DISCONNECTED;
      end
      Expected_ASC_Prep_Flag = false;
      Expected_Chrgr_Prep_Flag = false;
      Expected_PrechgVoltFlt = false;
      verify(AppOut_BMSMODE == Expected_BMSMODE );
      verify(AppOut_PrechgMosfet == Expected_PrechgMosfet);
      verify(AppOut_HVMosfet == Expected_HVMosfet);
      verify(AppOut_DCDCMosfet == Expected_DCDCMosfet);
      verify(AppOut_ASC_Prep_Flag == Expected_ASC_Prep_Flag);
      verify(AppOut_Chrgr_Prep_Flag == Expected_Chrgr_Prep_Flag);
      verify(AppOut_PrechgVoltFlt == Expected_PrechgVoltFlt);
    (default) -> ChargeSequenceIgOff.step_1
  state ChargeSequenceIgOn
    state step_1
      if t < 0.2
      Expected_BMSMODE  = BMS_MODE_E.BMS_SLEEP;
      elseif t >= 0.2 && t < 0.4
      Expected_BMSMODE  = BMS_MODE_E.BMS_STANDBY;
      else
      Expected_BMSMODE  = BMS_MODE_E.BMS_CHARGE;
      end
      if t < 0.8
      Expected_PrechgMosfet = BMS_PMosfet_STS_E.PDISCONNECTED;
      elseif t >= 0.8 && t < 1.9
      Expected_PrechgMosfet = BMS_PMosfet_STS_E.PCONNECTED;
      else
      Expected_PrechgMosfet = BMS_PMosfet_STS_E.PDISCONNECTED;
      end
      if t < 1.3
      Expected_HVMosfet = BMS_HVMosfet_STS_E.HV_DISCONNECTED;
      elseif t >= 1.3 && t < 1.9
      Expected_HVMosfet = BMS_HVMosfet_STS_E.HV_CONNECT_PENDING;
      else
      Expected_HVMosfet = BMS_HVMosfet_STS_E.HV_CONNECTED;
      end
      if t < 1.6
      Expected_DCDCMosfet = BMS_DCDCMosfet_STS_E.DCDC_DISCONNECTED;
      elseif t >= 1.6 && t < 3
      Expected_DCDCMosfet = BMS_DCDCMosfet_STS_E.DCDC_CONNECTED;
      elseif t >= 3 && t < 3.3
      Expected_DCDCMosfet = BMS_DCDCMosfet_STS_E.DCDC_DISCONNECTED;
      else
      Expected_DCDCMosfet = BMS_DCDCMosfet_STS_E.DCDC_CONNECTED;
      end
      Expected_ASC_Prep_Flag = false;
      Expected_Chrgr_Prep_Flag = false;
      Expected_PrechgVoltFlt = false;
      verify(AppOut_BMSMODE == Expected_BMSMODE );
      verify(AppOut_PrechgMosfet == Expected_PrechgMosfet);
      verify(AppOut_HVMosfet == Expected_HVMosfet);
      verify(AppOut_DCDCMosfet == Expected_DCDCMosfet);
      verify(AppOut_ASC_Prep_Flag == Expected_ASC_Prep_Flag);
      verify(AppOut_Chrgr_Prep_Flag == Expected_Chrgr_Prep_Flag);
      verify(AppOut_PrechgVoltFlt == Expected_PrechgVoltFlt);
    (default) -> ChargeSequenceIgOn.step_1
  state DischgToChargeAndIgOnToOff
    state step_1
      if t < 0.2
      Expected_BMSMODE  = BMS_MODE_E.BMS_SLEEP;
      elseif t >= 0.2 && t < 0.4
      Expected_BMSMODE  = BMS_MODE_E.BMS_STANDBY;
      elseif t >= 0.4 && t < 3
      Expected_BMSMODE  = BMS_MODE_E.BMS_DISCHARGE;
      elseif t >= 3 && t < 3.1
      Expected_BMSMODE  = BMS_MODE_E.BMS_STANDBY;
      else
      Expected_BMSMODE  = BMS_MODE_E.BMS_CHARGE;
      end
      if t < 0.8
      Expected_PrechgMosfet = BMS_PMosfet_STS_E.PDISCONNECTED;
      elseif t >= 0.8 && t < 1.9
      Expected_PrechgMosfet = BMS_PMosfet_STS_E.PCONNECTED;
      else
      Expected_PrechgMosfet = BMS_PMosfet_STS_E.PDISCONNECTED;
      end
      if t < 1.3
      Expected_HVMosfet = BMS_HVMosfet_STS_E.HV_DISCONNECTED;
      elseif t >= 1.3 && t < 1.9
      Expected_HVMosfet = BMS_HVMosfet_STS_E.HV_CONNECT_PENDING;
      else
      Expected_HVMosfet = BMS_HVMosfet_STS_E.HV_CONNECTED;
      end
      if t < 1.6
      Expected_DCDCMosfet = BMS_DCDCMosfet_STS_E.DCDC_DISCONNECTED;
      elseif t >= 1.6 && t < 4.5
      Expected_DCDCMosfet = BMS_DCDCMosfet_STS_E.DCDC_CONNECTED;
      else
      Expected_DCDCMosfet = BMS_DCDCMosfet_STS_E.DCDC_DISCONNECTED;
      end
      Expected_ASC_Prep_Flag = false;
      Expected_Chrgr_Prep_Flag = false;
      Expected_PrechgVoltFlt = false;
      verify(AppOut_BMSMODE == Expected_BMSMODE );
      verify(AppOut_PrechgMosfet == Expected_PrechgMosfet);
      verify(AppOut_HVMosfet == Expected_HVMosfet);
      verify(AppOut_DCDCMosfet == Expected_DCDCMosfet);
      verify(AppOut_ASC_Prep_Flag == Expected_ASC_Prep_Flag);
      verify(AppOut_Chrgr_Prep_Flag == Expected_Chrgr_Prep_Flag);
      verify(AppOut_PrechgVoltFlt == Expected_PrechgVoltFlt);
    (default) -> DischgToChargeAndIgOnToOff.step_1
  state G4T2DischargeToSleep
    state step_1
      if t < 0.2
      Expected_BMSMODE  = BMS_MODE_E.BMS_SLEEP;
      elseif t >= 0.2 && t < 0.4
      Expected_BMSMODE  = BMS_MODE_E.BMS_STANDBY;
      elseif t >= 0.4 && t < 3
      Expected_BMSMODE  = BMS_MODE_E.BMS_DISCHARGE;
      elseif t >= 3 && t < 13
      Expected_BMSMODE  = BMS_MODE_E.BMS_FAULT;
      else
      Expected_BMSMODE  = BMS_MODE_E.BMS_SLEEP;
      end
      if t < 0.8
      Expected_PrechgMosfet = BMS_PMosfet_STS_E.PDISCONNECTED;
      elseif t >= 0.8 && t < 1.9
      Expected_PrechgMosfet = BMS_PMosfet_STS_E.PCONNECTED;
      else
      Expected_PrechgMosfet = BMS_PMosfet_STS_E.PDISCONNECTED;
      end
      if t < 1.3
      Expected_HVMosfet = BMS_HVMosfet_STS_E.HV_DISCONNECTED;
      elseif t >= 1.3 && t < 1.9
      Expected_HVMosfet = BMS_HVMosfet_STS_E.HV_CONNECT_PENDING;
      elseif t >= 1.9 && t < 8.1
      Expected_HVMosfet = BMS_HVMosfet_STS_E.HV_CONNECTED;
      else
      Expected_HVMosfet = BMS_HVMosfet_STS_E.HV_DISCONNECTED;
      end
      if t < 1.6
      Expected_DCDCMosfet = BMS_DCDCMosfet_STS_E.DCDC_DISCONNECTED;
      elseif t >= 1.6 && t < 8.1
      Expected_DCDCMosfet = BMS_DCDCMosfet_STS_E.DCDC_CONNECTED;
      else
      Expected_DCDCMosfet = BMS_DCDCMosfet_STS_E.DCDC_DISCONNECTED;
      end
      if t < 3
      Expected_ASC_Prep_Flag = false;
      elseif t >= 3 && t < 8.1
      Expected_ASC_Prep_Flag = true;
      else
      Expected_ASC_Prep_Flag = false;
      end
      Expected_Chrgr_Prep_Flag = false;
      Expected_PrechgVoltFlt = false;
      verify(AppOut_BMSMODE == Expected_BMSMODE );
      verify(AppOut_PrechgMosfet == Expected_PrechgMosfet);
      verify(AppOut_HVMosfet == Expected_HVMosfet);
      verify(AppOut_DCDCMosfet == Expected_DCDCMosfet);
      verify(AppOut_ASC_Prep_Flag == Expected_ASC_Prep_Flag);
      verify(AppOut_Chrgr_Prep_Flag == Expected_Chrgr_Prep_Flag);
      verify(AppOut_PrechgVoltFlt == Expected_PrechgVoltFlt);
    (default) -> G4T2DischargeToSleep.step_1
  state G4Typ2DischgToSleep
    state step_1
      if t < 0.2
      Expected_BMSMODE  = BMS_MODE_E.BMS_SLEEP;
      elseif t >= 0.2 && t < 0.4
      Expected_BMSMODE  = BMS_MODE_E.BMS_STANDBY;
      elseif t >= 0.4 && t < 3
      Expected_BMSMODE  = BMS_MODE_E.BMS_DISCHARGE;
      elseif t >= 3 && t < 13
      Expected_BMSMODE  = BMS_MODE_E.BMS_FAULT;
      else
      Expected_BMSMODE  = BMS_MODE_E.BMS_SLEEP;
      end
      if t < 0.8
      Expected_PrechgMosfet = BMS_PMosfet_STS_E.PDISCONNECTED;
      elseif t >= 0.8 && t < 1.9
      Expected_PrechgMosfet = BMS_PMosfet_STS_E.PCONNECTED;
      else
      Expected_PrechgMosfet = BMS_PMosfet_STS_E.PDISCONNECTED;
      end
      if t < 1.3
      Expected_HVMosfet = BMS_HVMosfet_STS_E.HV_DISCONNECTED;
      elseif t >= 1.3 && t < 1.9
      Expected_HVMosfet = BMS_HVMosfet_STS_E.HV_CONNECT_PENDING;
      elseif t >= 1.9 && t < 8.1
      Expected_HVMosfet = BMS_HVMosfet_STS_E.HV_CONNECTED;
      else
      Expected_HVMosfet = BMS_HVMosfet_STS_E.HV_DISCONNECTED;
      end
      if t < 1.6
      Expected_DCDCMosfet = BMS_DCDCMosfet_STS_E.DCDC_DISCONNECTED;
      elseif t >= 1.6 && t < 8.1
      Expected_DCDCMosfet = BMS_DCDCMosfet_STS_E.DCDC_CONNECTED;
      else
      Expected_DCDCMosfet = BMS_DCDCMosfet_STS_E.DCDC_DISCONNECTED;
      end
      if t < 3
      Expected_ASC_Prep_Flag = false;
      elseif t >= 3 && t < 8.1
      Expected_ASC_Prep_Flag = true;
      else
      Expected_ASC_Prep_Flag = false;
      end
      Expected_Chrgr_Prep_Flag = false;
      Expected_PrechgVoltFlt = false;
      verify(AppOut_BMSMODE == Expected_BMSMODE );
      verify(AppOut_PrechgMosfet == Expected_PrechgMosfet);
      verify(AppOut_HVMosfet == Expected_HVMosfet);
      verify(AppOut_DCDCMosfet == Expected_DCDCMosfet);
      verify(AppOut_ASC_Prep_Flag == Expected_ASC_Prep_Flag);
      verify(AppOut_Chrgr_Prep_Flag == Expected_Chrgr_Prep_Flag);
      verify(AppOut_PrechgVoltFlt == Expected_PrechgVoltFlt);
    (default) -> G4Typ2DischgToSleep.step_1
  state G4T1DischargeToSleep
    state step_1
      if t < 0.2
      Expected_BMSMODE  = BMS_MODE_E.BMS_SLEEP;
      elseif t >= 0.2 && t < 0.4
      Expected_BMSMODE  = BMS_MODE_E.BMS_STANDBY;
      elseif t >= 0.4 && t < 3
      Expected_BMSMODE  = BMS_MODE_E.BMS_DISCHARGE;
      elseif t >= 3 && t < 13
      Expected_BMSMODE  = BMS_MODE_E.BMS_FAULT;
      else
      Expected_BMSMODE  = BMS_MODE_E.BMS_SLEEP;
      end
      if t < 0.8
      Expected_PrechgMosfet = BMS_PMosfet_STS_E.PDISCONNECTED;
      elseif t >= 0.8 && t < 1.9
      Expected_PrechgMosfet = BMS_PMosfet_STS_E.PCONNECTED;
      else
      Expected_PrechgMosfet = BMS_PMosfet_STS_E.PDISCONNECTED;
      end
      if t < 1.3
      Expected_HVMosfet = BMS_HVMosfet_STS_E.HV_DISCONNECTED;
      elseif t >= 1.3 && t < 1.9
      Expected_HVMosfet = BMS_HVMosfet_STS_E.HV_CONNECT_PENDING;
      elseif t >= 1.9 && t < 8.1
      Expected_HVMosfet = BMS_HVMosfet_STS_E.HV_CONNECTED;
      else
      Expected_HVMosfet = BMS_HVMosfet_STS_E.HV_DISCONNECTED;
      end
      if t < 1.6
      Expected_DCDCMosfet = BMS_DCDCMosfet_STS_E.DCDC_DISCONNECTED;
      elseif t >= 1.6 && t < 13
      Expected_DCDCMosfet = BMS_DCDCMosfet_STS_E.DCDC_CONNECTED;
      else
      Expected_DCDCMosfet = BMS_DCDCMosfet_STS_E.DCDC_DISCONNECTED;
      end
      if t < 3
      Expected_ASC_Prep_Flag = false;
      elseif t >= 3 && t < 8.1
      Expected_ASC_Prep_Flag = true;
      else
      Expected_ASC_Prep_Flag = false;
      end
      Expected_Chrgr_Prep_Flag = false;
      Expected_PrechgVoltFlt = false;
      verify(AppOut_BMSMODE == Expected_BMSMODE );
      verify(AppOut_PrechgMosfet == Expected_PrechgMosfet);
      verify(AppOut_HVMosfet == Expected_HVMosfet);
      verify(AppOut_DCDCMosfet == Expected_DCDCMosfet);
      verify(AppOut_ASC_Prep_Flag == Expected_ASC_Prep_Flag);
      verify(AppOut_Chrgr_Prep_Flag == Expected_Chrgr_Prep_Flag);
      verify(AppOut_PrechgVoltFlt == Expected_PrechgVoltFlt);
    (default) -> G4T1DischargeToSleep.step_1
  state G4Typ1DischgToSleep
    state step_1
      if t < 0.2
      Expected_BMSMODE  = BMS_MODE_E.BMS_SLEEP;
      elseif t >= 0.2 && t < 0.4
      Expected_BMSMODE  = BMS_MODE_E.BMS_STANDBY;
      elseif t >= 0.4 && t < 3
      Expected_BMSMODE  = BMS_MODE_E.BMS_DISCHARGE;
      elseif t >= 3 && t < 13
      Expected_BMSMODE  = BMS_MODE_E.BMS_FAULT;
      else
      Expected_BMSMODE  = BMS_MODE_E.BMS_SLEEP;
      end
      if t < 0.8
      Expected_PrechgMosfet = BMS_PMosfet_STS_E.PDISCONNECTED;
      elseif t >= 0.8 && t < 1.9
      Expected_PrechgMosfet = BMS_PMosfet_STS_E.PCONNECTED;
      else
      Expected_PrechgMosfet = BMS_PMosfet_STS_E.PDISCONNECTED;
      end
      if t < 1.3
      Expected_HVMosfet = BMS_HVMosfet_STS_E.HV_DISCONNECTED;
      elseif t >= 1.3 && t < 1.9
      Expected_HVMosfet = BMS_HVMosfet_STS_E.HV_CONNECT_PENDING;
      elseif t >= 1.9 && t < 8.1
      Expected_HVMosfet = BMS_HVMosfet_STS_E.HV_CONNECTED;
      else
      Expected_HVMosfet = BMS_HVMosfet_STS_E.HV_DISCONNECTED;
      end
      if t < 1.6
      Expected_DCDCMosfet = BMS_DCDCMosfet_STS_E.DCDC_DISCONNECTED;
      elseif t >= 1.6 && t < 9
      Expected_DCDCMosfet = BMS_DCDCMosfet_STS_E.DCDC_CONNECTED;
      else
      Expected_DCDCMosfet = BMS_DCDCMosfet_STS_E.DCDC_DISCONNECTED;
      end
      if t < 3
      Expected_ASC_Prep_Flag = false;
      elseif t >= 3 && t < 8.1
      Expected_ASC_Prep_Flag = true;
      else
      Expected_ASC_Prep_Flag = false;
      end
      Expected_Chrgr_Prep_Flag = false;
      Expected_PrechgVoltFlt = false;
      verify(AppOut_BMSMODE == Expected_BMSMODE );
      verify(AppOut_PrechgMosfet == Expected_PrechgMosfet);
      verify(AppOut_HVMosfet == Expected_HVMosfet);
      verify(AppOut_DCDCMosfet == Expected_DCDCMosfet);
      verify(AppOut_ASC_Prep_Flag == Expected_ASC_Prep_Flag);
      verify(AppOut_Chrgr_Prep_Flag == Expected_Chrgr_Prep_Flag);
      verify(AppOut_PrechgVoltFlt == Expected_PrechgVoltFlt);
    (default) -> G4Typ1DischgToSleep.step_1
  state G4CommonToSleep
    state step_1
      if t < 0.2
      Expected_BMSMODE  = BMS_MODE_E.BMS_SLEEP;
      elseif t >= 0.2 && t < 0.4
      Expected_BMSMODE  = BMS_MODE_E.BMS_STANDBY;
      elseif t >= 0.4 && t < 3
      Expected_BMSMODE  = BMS_MODE_E.BMS_DISCHARGE;
      elseif t >= 3 && t < 13
      Expected_BMSMODE  = BMS_MODE_E.BMS_FAULT;
      else
      Expected_BMSMODE  = BMS_MODE_E.BMS_SLEEP;
      end
      if t < 0.8
      Expected_PrechgMosfet = BMS_PMosfet_STS_E.PDISCONNECTED;
      elseif t >= 0.8 && t < 1.9
      Expected_PrechgMosfet = BMS_PMosfet_STS_E.PCONNECTED;
      else
      Expected_PrechgMosfet = BMS_PMosfet_STS_E.PDISCONNECTED;
      end
      if t < 1.3
      Expected_HVMosfet = BMS_HVMosfet_STS_E.HV_DISCONNECTED;
      elseif t >= 1.3 && t < 1.9
      Expected_HVMosfet = BMS_HVMosfet_STS_E.HV_CONNECT_PENDING;
      elseif t >= 1.9 && t < 8.1
      Expected_HVMosfet = BMS_HVMosfet_STS_E.HV_CONNECTED;
      else
      Expected_HVMosfet = BMS_HVMosfet_STS_E.HV_DISCONNECTED;
      end
      if t < 1.6
      Expected_DCDCMosfet = BMS_DCDCMosfet_STS_E.DCDC_DISCONNECTED;
      elseif t >= 1.6 && t < 13
      Expected_DCDCMosfet = BMS_DCDCMosfet_STS_E.DCDC_CONNECTED;
      else
      Expected_DCDCMosfet = BMS_DCDCMosfet_STS_E.DCDC_DISCONNECTED;
      end
      if t < 3
      Expected_ASC_Prep_Flag = false;
      elseif t >= 3 && t < 8.1
      Expected_ASC_Prep_Flag = true;
      else
      Expected_ASC_Prep_Flag = false;
      end
      if t < 3
      Expected_Chrgr_Prep_Flag = false;
      elseif t >= 3 && t < 8.1
      Expected_Chrgr_Prep_Flag = true;
      else
      Expected_Chrgr_Prep_Flag = false;
      end
      Expected_PrechgVoltFlt = false;
      verify(AppOut_BMSMODE == Expected_BMSMODE );
      verify(AppOut_PrechgMosfet == Expected_PrechgMosfet);
      verify(AppOut_HVMosfet == Expected_HVMosfet);
      verify(AppOut_DCDCMosfet == Expected_DCDCMosfet);
      verify(AppOut_ASC_Prep_Flag == Expected_ASC_Prep_Flag);
      verify(AppOut_Chrgr_Prep_Flag == Expected_Chrgr_Prep_Flag);
      verify(AppOut_PrechgVoltFlt == Expected_PrechgVoltFlt);
    (default) -> G4CommonToSleep.step_1
  state G4CommToSleep
    state step_1
      if t < 0.2
      Expected_BMSMODE  = BMS_MODE_E.BMS_SLEEP;
      elseif t >= 0.2 && t < 0.4
      Expected_BMSMODE  = BMS_MODE_E.BMS_STANDBY;
      elseif t >= 0.4 && t < 3
      Expected_BMSMODE  = BMS_MODE_E.BMS_DISCHARGE;
      elseif t >= 3 && t < 13
      Expected_BMSMODE  = BMS_MODE_E.BMS_FAULT;
      else
      Expected_BMSMODE  = BMS_MODE_E.BMS_SLEEP;
      end
      if t < 0.8
      Expected_PrechgMosfet = BMS_PMosfet_STS_E.PDISCONNECTED;
      elseif t >= 0.8 && t < 1.9
      Expected_PrechgMosfet = BMS_PMosfet_STS_E.PCONNECTED;
      else
      Expected_PrechgMosfet = BMS_PMosfet_STS_E.PDISCONNECTED;
      end
      if t < 1.3
      Expected_HVMosfet = BMS_HVMosfet_STS_E.HV_DISCONNECTED;
      elseif t >= 1.3 && t < 1.9
      Expected_HVMosfet = BMS_HVMosfet_STS_E.HV_CONNECT_PENDING;
      elseif t >= 1.9 && t < 8.1
      Expected_HVMosfet = BMS_HVMosfet_STS_E.HV_CONNECTED;
      else
      Expected_HVMosfet = BMS_HVMosfet_STS_E.HV_DISCONNECTED;
      end
      if t < 1.6
      Expected_DCDCMosfet = BMS_DCDCMosfet_STS_E.DCDC_DISCONNECTED;
      elseif t >= 1.6 && t < 9.1
      Expected_DCDCMosfet = BMS_DCDCMosfet_STS_E.DCDC_CONNECTED;
      else
      Expected_DCDCMosfet = BMS_DCDCMosfet_STS_E.DCDC_DISCONNECTED;
      end
      if t < 3
      Expected_ASC_Prep_Flag = false;
      elseif t >= 3 && t < 8.1
      Expected_ASC_Prep_Flag = true;
      else
      Expected_ASC_Prep_Flag = false;
      end
      if t < 3
      Expected_Chrgr_Prep_Flag = false;
      elseif t >= 3 && t < 8.1
      Expected_Chrgr_Prep_Flag = true;
      else
      Expected_Chrgr_Prep_Flag = false;
      end
      Expected_PrechgVoltFlt = false;
      verify(AppOut_BMSMODE == Expected_BMSMODE );
      verify(AppOut_PrechgMosfet == Expected_PrechgMosfet);
      verify(AppOut_HVMosfet == Expected_HVMosfet);
      verify(AppOut_DCDCMosfet == Expected_DCDCMosfet);
      verify(AppOut_ASC_Prep_Flag == Expected_ASC_Prep_Flag);
      verify(AppOut_Chrgr_Prep_Flag == Expected_Chrgr_Prep_Flag);
      verify(AppOut_PrechgVoltFlt == Expected_PrechgVoltFlt);
    (default) -> G4CommToSleep.step_1
  state G4ChargeToSleep
    state step_1
      if t < 0.2
      Expected_BMSMODE  = BMS_MODE_E.BMS_SLEEP;
      elseif t >= 0.2 && t < 0.4
      Expected_BMSMODE  = BMS_MODE_E.BMS_STANDBY;
      elseif t >= 0.4 && t < 3
      Expected_BMSMODE  = BMS_MODE_E.BMS_CHARGE;
      elseif t >= 3 && t < 13
      Expected_BMSMODE  = BMS_MODE_E.BMS_FAULT;
      else
      Expected_BMSMODE  = BMS_MODE_E.BMS_SLEEP;
      end
      if t < 0.8
      Expected_PrechgMosfet = BMS_PMosfet_STS_E.PDISCONNECTED;
      elseif t >= 0.8 && t < 1.9
      Expected_PrechgMosfet = BMS_PMosfet_STS_E.PCONNECTED;
      else
      Expected_PrechgMosfet = BMS_PMosfet_STS_E.PDISCONNECTED;
      end
      if t < 1.3
      Expected_HVMosfet = BMS_HVMosfet_STS_E.HV_DISCONNECTED;
      elseif t >= 1.3 && t < 1.9
      Expected_HVMosfet = BMS_HVMosfet_STS_E.HV_CONNECT_PENDING;
      elseif t >= 1.9 && t < 8.1
      Expected_HVMosfet = BMS_HVMosfet_STS_E.HV_CONNECTED;
      else
      Expected_HVMosfet = BMS_HVMosfet_STS_E.HV_DISCONNECTED;
      end
      if t < 1.6
      Expected_DCDCMosfet = BMS_DCDCMosfet_STS_E.DCDC_DISCONNECTED;
      elseif t >= 1.6 && t < 13
      Expected_DCDCMosfet = BMS_DCDCMosfet_STS_E.DCDC_CONNECTED;
      else
      Expected_DCDCMosfet = BMS_DCDCMosfet_STS_E.DCDC_DISCONNECTED;
      end
      Expected_ASC_Prep_Flag = false;
      if t < 3
      Expected_Chrgr_Prep_Flag = false;
      elseif t >= 3 && t < 8.1
      Expected_Chrgr_Prep_Flag = true;
      else
      Expected_Chrgr_Prep_Flag = false;
      end
      Expected_PrechgVoltFlt = false;
      verify(AppOut_BMSMODE == Expected_BMSMODE );
      verify(AppOut_PrechgMosfet == Expected_PrechgMosfet);
      verify(AppOut_HVMosfet == Expected_HVMosfet);
      verify(AppOut_DCDCMosfet == Expected_DCDCMosfet);
      verify(AppOut_ASC_Prep_Flag == Expected_ASC_Prep_Flag);
      verify(AppOut_Chrgr_Prep_Flag == Expected_Chrgr_Prep_Flag);
      verify(AppOut_PrechgVoltFlt == Expected_PrechgVoltFlt);
    (default) -> G4ChargeToSleep.step_1
  state G4ChgToSleep
    state step_1
      if t < 0.2
      Expected_BMSMODE  = BMS_MODE_E.BMS_SLEEP;
      elseif t >= 0.2 && t < 0.4
      Expected_BMSMODE  = BMS_MODE_E.BMS_STANDBY;
      elseif t >= 0.4 && t < 3
      Expected_BMSMODE  = BMS_MODE_E.BMS_CHARGE;
      elseif t >= 3 && t < 13
      Expected_BMSMODE  = BMS_MODE_E.BMS_FAULT;
      else
      Expected_BMSMODE  = BMS_MODE_E.BMS_SLEEP;
      end
      if t < 0.8
      Expected_PrechgMosfet = BMS_PMosfet_STS_E.PDISCONNECTED;
      elseif t >= 0.8 && t < 1.9
      Expected_PrechgMosfet = BMS_PMosfet_STS_E.PCONNECTED;
      else
      Expected_PrechgMosfet = BMS_PMosfet_STS_E.PDISCONNECTED;
      end
      if t < 1.3
      Expected_HVMosfet = BMS_HVMosfet_STS_E.HV_DISCONNECTED;
      elseif t >= 1.3 && t < 1.9
      Expected_HVMosfet = BMS_HVMosfet_STS_E.HV_CONNECT_PENDING;
      elseif t >= 1.9 && t < 8.1
      Expected_HVMosfet = BMS_HVMosfet_STS_E.HV_CONNECTED;
      else
      Expected_HVMosfet = BMS_HVMosfet_STS_E.HV_DISCONNECTED;
      end
      if t < 1.6
      Expected_DCDCMosfet = BMS_DCDCMosfet_STS_E.DCDC_DISCONNECTED;
      elseif t >= 1.6 && t < 9
      Expected_DCDCMosfet = BMS_DCDCMosfet_STS_E.DCDC_CONNECTED;
      else
      Expected_DCDCMosfet = BMS_DCDCMosfet_STS_E.DCDC_DISCONNECTED;
      end
      Expected_ASC_Prep_Flag = false;
      if t < 3
      Expected_Chrgr_Prep_Flag = false;
      elseif t >= 3 && t < 8.1
      Expected_Chrgr_Prep_Flag = true;
      else
      Expected_Chrgr_Prep_Flag = false;
      end
      Expected_PrechgVoltFlt = false;
      verify(AppOut_BMSMODE == Expected_BMSMODE );
      verify(AppOut_PrechgMosfet == Expected_PrechgMosfet);
      verify(AppOut_HVMosfet == Expected_HVMosfet);
      verify(AppOut_DCDCMosfet == Expected_DCDCMosfet);
      verify(AppOut_ASC_Prep_Flag == Expected_ASC_Prep_Flag);
      verify(AppOut_Chrgr_Prep_Flag == Expected_Chrgr_Prep_Flag);
      verify(AppOut_PrechgVoltFlt == Expected_PrechgVoltFlt);
    (default) -> G4ChgToSleep.step_1
  state ChgToDischgToSleep
    state step_1
      if t < 0.2
      Expected_BMSMODE  = BMS_MODE_E.BMS_SLEEP;
      elseif t >= 0.2 && t < 0.4
      Expected_BMSMODE  = BMS_MODE_E.BMS_STANDBY;
      elseif t >= 0.4 && t < 4.1
      Expected_BMSMODE  = BMS_MODE_E.BMS_CHARGE;
      elseif t >= 4.1 && t < 4.3
      Expected_BMSMODE  = BMS_MODE_E.BMS_STANDBY;
      elseif t >= 4.3 && t < 4.8
      Expected_BMSMODE  = BMS_MODE_E.BMS_DISCHARGE;
      elseif t >= 4.8 && t < 14.8
      Expected_BMSMODE  = BMS_MODE_E.BMS_STANDBY;
      else
      Expected_BMSMODE  = BMS_MODE_E.BMS_SLEEP;
      end
      if t < 1.1
      Expected_PrechgMosfet = BMS_PMosfet_STS_E.PDISCONNECTED;
      elseif t >= 1.1 && t < 2.8
      Expected_PrechgMosfet = BMS_PMosfet_STS_E.PCONNECTED;
      else
      Expected_PrechgMosfet = BMS_PMosfet_STS_E.PDISCONNECTED;
      end
      if t < 1.8
      Expected_HVMosfet = BMS_HVMosfet_STS_E.HV_DISCONNECTED;
      elseif t >= 1.8 && t < 2.8
      Expected_HVMosfet = BMS_HVMosfet_STS_E.HV_CONNECT_PENDING;
      elseif t >= 2.8 && t < 5
      Expected_HVMosfet = BMS_HVMosfet_STS_E.HV_CONNECTED;
      else
      Expected_HVMosfet = BMS_HVMosfet_STS_E.HV_DISCONNECTED;
      end
      if t < 2.3
      Expected_DCDCMosfet = BMS_DCDCMosfet_STS_E.DCDC_DISCONNECTED;
      elseif t >= 2.3 && t < 14.8
      Expected_DCDCMosfet = BMS_DCDCMosfet_STS_E.DCDC_CONNECTED;
      else
      Expected_DCDCMosfet = BMS_DCDCMosfet_STS_E.DCDC_DISCONNECTED;
      end
      Expected_ASC_Prep_Flag = false;
      Expected_Chrgr_Prep_Flag = false;
      Expected_PrechgVoltFlt = false;
      verify(AppOut_BMSMODE == Expected_BMSMODE );
      verify(AppOut_PrechgMosfet == Expected_PrechgMosfet);
      verify(AppOut_HVMosfet == Expected_HVMosfet);
      verify(AppOut_DCDCMosfet == Expected_DCDCMosfet);
      verify(AppOut_ASC_Prep_Flag == Expected_ASC_Prep_Flag);
      verify(AppOut_Chrgr_Prep_Flag == Expected_Chrgr_Prep_Flag);
      verify(AppOut_PrechgVoltFlt == Expected_PrechgVoltFlt);
    (default) -> ChgToDischgToSleep.step_1
  state G4CommToChg
    state step_1
      if t < 0.2
      Expected_BMSMODE  = BMS_MODE_E.BMS_SLEEP;
      elseif t >= 0.2 && t < 0.4
      Expected_BMSMODE  = BMS_MODE_E.BMS_STANDBY;
      elseif t >= 0.4 && t < 3
      Expected_BMSMODE  = BMS_MODE_E.BMS_DISCHARGE;
      elseif t >= 3 && t < 9.2
      Expected_BMSMODE  = BMS_MODE_E.BMS_FAULT;
      else
      Expected_BMSMODE  = BMS_MODE_E.BMS_CHARGE;
      end
      if t < 0.8
      Expected_PrechgMosfet = BMS_PMosfet_STS_E.PDISCONNECTED;
      elseif t >= 0.8 && t < 1.9
      Expected_PrechgMosfet = BMS_PMosfet_STS_E.PCONNECTED;
      elseif t >= 1.9 && t < 9.6
      Expected_PrechgMosfet = BMS_PMosfet_STS_E.PDISCONNECTED;
      elseif t >= 9.6 && t < 10.6
      Expected_PrechgMosfet = BMS_PMosfet_STS_E.PCONNECTED;
      else
      Expected_PrechgMosfet = BMS_PMosfet_STS_E.PDISCONNECTED;
      end
      if t < 1.3
      Expected_HVMosfet = BMS_HVMosfet_STS_E.HV_DISCONNECTED;
      elseif t >= 1.3 && t < 1.9
      Expected_HVMosfet = BMS_HVMosfet_STS_E.HV_CONNECT_PENDING;
      elseif t >= 1.9 && t < 8.1
      Expected_HVMosfet = BMS_HVMosfet_STS_E.HV_CONNECTED;
      elseif t >= 8.1 && t < 9.9
      Expected_HVMosfet = BMS_HVMosfet_STS_E.HV_DISCONNECTED;
      elseif t >= 9.9 && t < 10.6
      Expected_HVMosfet = BMS_HVMosfet_STS_E.HV_CONNECT_PENDING;
      else
      Expected_HVMosfet = BMS_HVMosfet_STS_E.HV_CONNECTED;
      end
      if t < 1.6
      Expected_DCDCMosfet = BMS_DCDCMosfet_STS_E.DCDC_DISCONNECTED;
      elseif t >= 1.6 && t < 10.3
      Expected_DCDCMosfet = BMS_DCDCMosfet_STS_E.DCDC_CONNECTED;
      else
      Expected_DCDCMosfet = BMS_DCDCMosfet_STS_E.DCDC_DISCONNECTED;
      end
      if t < 3
      Expected_ASC_Prep_Flag = false;
      elseif t >= 3 && t < 8.1
      Expected_ASC_Prep_Flag = true;
      else
      Expected_ASC_Prep_Flag = false;
      end
      if t < 3
      Expected_Chrgr_Prep_Flag = false;
      elseif t >= 3 && t < 8.1
      Expected_Chrgr_Prep_Flag = true;
      else
      Expected_Chrgr_Prep_Flag = false;
      end
      Expected_PrechgVoltFlt = false;
      verify(AppOut_BMSMODE == Expected_BMSMODE );
      verify(AppOut_PrechgMosfet == Expected_PrechgMosfet);
      verify(AppOut_HVMosfet == Expected_HVMosfet);
      verify(AppOut_DCDCMosfet == Expected_DCDCMosfet);
      verify(AppOut_ASC_Prep_Flag == Expected_ASC_Prep_Flag);
      verify(AppOut_Chrgr_Prep_Flag == Expected_Chrgr_Prep_Flag);
      verify(AppOut_PrechgVoltFlt == Expected_PrechgVoltFlt);
    (default) -> G4CommToChg.step_1
  state G4ChgFltToDischg
    state step_1
      if t < 0.2
      Expected_BMSMODE  = BMS_MODE_E.BMS_SLEEP;
      elseif t >= 0.2 && t < 0.3
      Expected_BMSMODE  = BMS_MODE_E.BMS_STANDBY;
      elseif t >= 0.3 && t < 2.7
      Expected_BMSMODE  = BMS_MODE_E.BMS_CHARGE;
      elseif t >= 2.7 && t < 8.7
      Expected_BMSMODE  = BMS_MODE_E.BMS_FAULT;
      else
      Expected_BMSMODE  = BMS_MODE_E.BMS_DISCHARGE;
      end
      if t < 0.6
      Expected_PrechgMosfet = BMS_PMosfet_STS_E.PDISCONNECTED;
      elseif t >= 0.6 && t < 1.6
      Expected_PrechgMosfet = BMS_PMosfet_STS_E.PCONNECTED;
      elseif t >= 1.6 && t < 9.1
      Expected_PrechgMosfet = BMS_PMosfet_STS_E.PDISCONNECTED;
      elseif t >= 9.1 && t < 10
      Expected_PrechgMosfet = BMS_PMosfet_STS_E.PCONNECTED;
      else
      Expected_PrechgMosfet = BMS_PMosfet_STS_E.PDISCONNECTED;
      end
      if t < 1.1
      Expected_HVMosfet = BMS_HVMosfet_STS_E.HV_DISCONNECTED;
      elseif t >= 1.1 && t < 1.6
      Expected_HVMosfet = BMS_HVMosfet_STS_E.HV_CONNECT_PENDING;
      elseif t >= 1.6 && t < 7.8
      Expected_HVMosfet = BMS_HVMosfet_STS_E.HV_CONNECTED;
      elseif t >= 7.8 && t < 9.4
      Expected_HVMosfet = BMS_HVMosfet_STS_E.HV_DISCONNECTED;
      elseif t >= 9.4 && t < 10
      Expected_HVMosfet = BMS_HVMosfet_STS_E.HV_CONNECT_PENDING;
      else
      Expected_HVMosfet = BMS_HVMosfet_STS_E.HV_CONNECTED;
      end
      if t < 9.7
      Expected_DCDCMosfet = BMS_DCDCMosfet_STS_E.DCDC_DISCONNECTED;
      else
      Expected_DCDCMosfet = BMS_DCDCMosfet_STS_E.DCDC_CONNECTED;
      end
      Expected_ASC_Prep_Flag = false;
      if t < 2.7
      Expected_Chrgr_Prep_Flag = false;
      elseif t >= 2.7 && t < 7.8
      Expected_Chrgr_Prep_Flag = true;
      else
      Expected_Chrgr_Prep_Flag = false;
      end
      Expected_PrechgVoltFlt = false;
      verify(AppOut_BMSMODE == Expected_BMSMODE );
      verify(AppOut_PrechgMosfet == Expected_PrechgMosfet);
      verify(AppOut_HVMosfet == Expected_HVMosfet);
      verify(AppOut_DCDCMosfet == Expected_DCDCMosfet);
      verify(AppOut_ASC_Prep_Flag == Expected_ASC_Prep_Flag);
      verify(AppOut_Chrgr_Prep_Flag == Expected_Chrgr_Prep_Flag);
      verify(AppOut_PrechgVoltFlt == Expected_PrechgVoltFlt);
    (default) -> G4ChgFltToDischg.step_1
  state G4T1DischgToG4T2Dischg
    state step_1
      if t < 0.2
      Expected_BMSMODE  = BMS_MODE_E.BMS_SLEEP;
      elseif t >= 0.2 && t < 0.4
      Expected_BMSMODE  = BMS_MODE_E.BMS_STANDBY;
      elseif t >= 0.4 && t < 3
      Expected_BMSMODE  = BMS_MODE_E.BMS_DISCHARGE;
      else
      Expected_BMSMODE  = BMS_MODE_E.BMS_FAULT;
      end
      if t < 0.8
      Expected_PrechgMosfet = BMS_PMosfet_STS_E.PDISCONNECTED;
      elseif t >= 0.8 && t < 1.9
      Expected_PrechgMosfet = BMS_PMosfet_STS_E.PCONNECTED;
      else
      Expected_PrechgMosfet = BMS_PMosfet_STS_E.PDISCONNECTED;
      end
      if t < 1.3
      Expected_HVMosfet = BMS_HVMosfet_STS_E.HV_DISCONNECTED;
      elseif t >= 1.3 && t < 1.9
      Expected_HVMosfet = BMS_HVMosfet_STS_E.HV_CONNECT_PENDING;
      elseif t >= 1.9 && t < 8.1
      Expected_HVMosfet = BMS_HVMosfet_STS_E.HV_CONNECTED;
      else
      Expected_HVMosfet = BMS_HVMosfet_STS_E.HV_DISCONNECTED;
      end
      if t < 1.6
      Expected_DCDCMosfet = BMS_DCDCMosfet_STS_E.DCDC_DISCONNECTED;
      elseif t >= 1.6 && t < 14.1
      Expected_DCDCMosfet = BMS_DCDCMosfet_STS_E.DCDC_CONNECTED;
      else
      Expected_DCDCMosfet = BMS_DCDCMosfet_STS_E.DCDC_DISCONNECTED;
      end
      if t < 3
      Expected_ASC_Prep_Flag = false;
      elseif t >= 3 && t < 8.1
      Expected_ASC_Prep_Flag = true;
      elseif t >= 8.1 && t < 9
      Expected_ASC_Prep_Flag = false;
      elseif t >= 9 && t < 14.1
      Expected_ASC_Prep_Flag = true;
      else
      Expected_ASC_Prep_Flag = false;
      end
      Expected_Chrgr_Prep_Flag = false;
      Expected_PrechgVoltFlt = false;
      verify(AppOut_BMSMODE == Expected_BMSMODE );
      verify(AppOut_PrechgMosfet == Expected_PrechgMosfet);
      verify(AppOut_HVMosfet == Expected_HVMosfet);
      verify(AppOut_DCDCMosfet == Expected_DCDCMosfet);
      verify(AppOut_ASC_Prep_Flag == Expected_ASC_Prep_Flag);
      verify(AppOut_Chrgr_Prep_Flag == Expected_Chrgr_Prep_Flag);
      verify(AppOut_PrechgVoltFlt == Expected_PrechgVoltFlt);
    (default) -> G4T1DischgToG4T2Dischg.step_1
  state SleepToCharge
    state step_1
      if t < 0.3
      Expected_BMSMODE  = BMS_MODE_E.BMS_SLEEP;
      elseif t >= 0.3 && t < 1.4
      Expected_BMSMODE  = BMS_MODE_E.BMS_STANDBY;
      elseif t >= 1.4 && t < 6.3
      Expected_BMSMODE  = BMS_MODE_E.BMS_CHARGE;
      elseif t >= 6.3 && t < 16.3
      Expected_BMSMODE  = BMS_MODE_E.BMS_STANDBY;
      else
      Expected_BMSMODE  = BMS_MODE_E.BMS_SLEEP;
      end
      verify(AppOut_BMSMODE == Expected_BMSMODE );
    (default) -> SleepToCharge.step_1
  state SleepToDischarge
    state step_1
      if t < 0.5
      Expected_BMSMODE  = BMS_MODE_E.BMS_SLEEP;
      elseif t >= 0.5 && t < 0.9
      Expected_BMSMODE  = BMS_MODE_E.BMS_STANDBY;
      elseif t >= 0.9 && t < 6.1
      Expected_BMSMODE  = BMS_MODE_E.BMS_DISCHARGE;
      elseif t >= 6.1 && t < 16.1
      Expected_BMSMODE  = BMS_MODE_E.BMS_STANDBY;
      else
      Expected_BMSMODE  = BMS_MODE_E.BMS_SLEEP;
      end
      verify(AppOut_BMSMODE == Expected_BMSMODE );
    (default) -> SleepToDischarge.step_1
  state SleepToChargeToSleep
    state step_1
      if t < 0.2
      Expected_BMSMODE  = BMS_MODE_E.BMS_SLEEP;
      elseif t >= 0.2 && t < 10.2
      Expected_BMSMODE  = BMS_MODE_E.BMS_STANDBY;
      elseif t >= 10.2 && t < 12.3
      Expected_BMSMODE  = BMS_MODE_E.BMS_SLEEP;
      elseif t >= 12.3 && t < 22.3
      Expected_BMSMODE  = BMS_MODE_E.BMS_STANDBY;
      else
      Expected_BMSMODE  = BMS_MODE_E.BMS_SLEEP;
      end
      verify(AppOut_BMSMODE == Expected_BMSMODE );
    (default) -> SleepToChargeToSleep.step_1
  state SleepToChg
    state step_1
      if t < 0.3
      Expected_BMSMODE  = BMS_MODE_E.BMS_SLEEP;
      elseif t >= 0.3 && t < 0.5
      Expected_BMSMODE  = BMS_MODE_E.BMS_STANDBY;
      elseif t >= 0.5 && t < 5.5
      Expected_BMSMODE  = BMS_MODE_E.BMS_CHARGE;
      elseif t >= 5.5 && t < 15.5
      Expected_BMSMODE  = BMS_MODE_E.BMS_STANDBY;
      else
      Expected_BMSMODE  = BMS_MODE_E.BMS_SLEEP;
      end
      verify(AppOut_BMSMODE == Expected_BMSMODE );
    (default) -> SleepToChg.step_1
  state SleepToChrg
    state step_1
      if t < 0.3
      Expected_BMSMODE  = BMS_MODE_E.BMS_SLEEP;
      elseif t >= 0.3 && t < 0.5
      Expected_BMSMODE  = BMS_MODE_E.BMS_STANDBY;
      elseif t >= 0.5 && t < 5.5
      Expected_BMSMODE  = BMS_MODE_E.BMS_CHARGE;
      elseif t >= 5.5 && t < 15.5
      Expected_BMSMODE  = BMS_MODE_E.BMS_STANDBY;
      else
      Expected_BMSMODE  = BMS_MODE_E.BMS_SLEEP;
      end
      verify(AppOut_BMSMODE == Expected_BMSMODE );
    (default) -> SleepToChrg.step_1
  state SleepToStbToG3CommFlt
    state step_1
      if t < 0.2
      Expected_BMSMODE  = BMS_MODE_E.BMS_SLEEP;
      elseif t >= 0.2 && t < 0.4
      Expected_BMSMODE  = BMS_MODE_E.BMS_STANDBY;
      elseif t >= 0.4 && t < 10.4
      Expected_BMSMODE  = BMS_MODE_E.BMS_FAULT;
      else
      Expected_BMSMODE  = BMS_MODE_E.BMS_SLEEP;
      end
      verify(AppOut_BMSMODE == Expected_BMSMODE );
    (default) -> SleepToStbToG3CommFlt.step_1
  state SleepToStbToG4CommFlt
    state step_1
      if t < 0.2
      Expected_BMSMODE  = BMS_MODE_E.BMS_SLEEP;
      elseif t >= 0.2 && t < 0.4
      Expected_BMSMODE  = BMS_MODE_E.BMS_STANDBY;
      elseif t >= 0.4 && t < 1.1
      Expected_BMSMODE  = BMS_MODE_E.BMS_FAULT;
      else
      Expected_BMSMODE  = BMS_MODE_E.BMS_SLEEP;
      end
      verify(AppOut_BMSMODE == Expected_BMSMODE );
    (default) -> SleepToStbToG4CommFlt.step_1
  state SleepToStbToG4CommFlt1
    state step_1
      if t < 0.2
      Expected_BMSMODE  = BMS_MODE_E.BMS_SLEEP;
      elseif t >= 0.2 && t < 0.4
      Expected_BMSMODE  = BMS_MODE_E.BMS_STANDBY;
      elseif t >= 0.4 && t < 1.1
      Expected_BMSMODE  = BMS_MODE_E.BMS_FAULT;
      elseif t >= 1.1 && t < 11.1
      Expected_BMSMODE  = BMS_MODE_E.BMS_STANDBY;
      else
      Expected_BMSMODE  = BMS_MODE_E.BMS_SLEEP;
      end
      verify(AppOut_BMSMODE == Expected_BMSMODE );
    (default) -> SleepToStbToG4CommFlt1.step_1
  state SleepToDischgToFlt
    state step_1
      if t < 0.2
      Expected_BMSMODE  = BMS_MODE_E.BMS_SLEEP;
      elseif t >= 0.2 && t < 0.4
      Expected_BMSMODE  = BMS_MODE_E.BMS_STANDBY;
      elseif t >= 0.4 && t < 2.4
      Expected_BMSMODE  = BMS_MODE_E.BMS_DISCHARGE;
      elseif t >= 2.4 && t < 8.4
      Expected_BMSMODE  = BMS_MODE_E.BMS_FAULT;
      elseif t >= 8.4 && t < 10.4
      Expected_BMSMODE  = BMS_MODE_E.BMS_DISCHARGE;
      elseif t >= 10.4 && t < 20.4
      Expected_BMSMODE  = BMS_MODE_E.BMS_STANDBY;
      else
      Expected_BMSMODE  = BMS_MODE_E.BMS_SLEEP;
      end
      verify(AppOut_BMSMODE == Expected_BMSMODE );
    (default) -> SleepToDischgToFlt.step_1
  state SleepToDischgToFlt1
    state step_1
      if t < 0.2
      Expected_BMSMODE  = BMS_MODE_E.BMS_SLEEP;
      elseif t >= 0.2 && t < 0.4
      Expected_BMSMODE  = BMS_MODE_E.BMS_STANDBY;
      elseif t >= 0.4 && t < 2.4
      Expected_BMSMODE  = BMS_MODE_E.BMS_DISCHARGE;
      elseif t >= 2.4 && t < 8.4
      Expected_BMSMODE  = BMS_MODE_E.BMS_FAULT;
      elseif t >= 8.4 && t < 10.4
      Expected_BMSMODE  = BMS_MODE_E.BMS_DISCHARGE;
      elseif t >= 10.4 && t < 20.4
      Expected_BMSMODE  = BMS_MODE_E.BMS_STANDBY;
      else
      Expected_BMSMODE  = BMS_MODE_E.BMS_SLEEP;
      end
      verify(AppOut_BMSMODE == Expected_BMSMODE );
    (default) -> SleepToDischgToFlt1.step_1
  state SleepToDischgToFlt2
    state step_1
      if t < 0.2
      Expected_BMSMODE  = BMS_MODE_E.BMS_SLEEP;
      elseif t >= 0.2 && t < 0.4
      Expected_BMSMODE  = BMS_MODE_E.BMS_STANDBY;
      elseif t >= 0.4 && t < 2.4
      Expected_BMSMODE  = BMS_MODE_E.BMS_DISCHARGE;
      elseif t >= 2.4 && t < 8.6
      Expected_BMSMODE  = BMS_MODE_E.BMS_FAULT;
      elseif t >= 8.6 && t < 10.6
      Expected_BMSMODE  = BMS_MODE_E.BMS_DISCHARGE;
      elseif t >= 10.6 && t < 20.6
      Expected_BMSMODE  = BMS_MODE_E.BMS_STANDBY;
      else
      Expected_BMSMODE  = BMS_MODE_E.BMS_SLEEP;
      end
      verify(AppOut_BMSMODE == Expected_BMSMODE );
    (default) -> SleepToDischgToFlt2.step_1
  state SleepToDischgToFlt3
    state step_1
      if t < 0.2
      Expected_BMSMODE  = BMS_MODE_E.BMS_SLEEP;
      elseif t >= 0.2 && t < 0.4
      Expected_BMSMODE  = BMS_MODE_E.BMS_STANDBY;
      elseif t >= 0.4 && t < 2.4
      Expected_BMSMODE  = BMS_MODE_E.BMS_DISCHARGE;
      elseif t >= 2.4 && t < 8.6
      Expected_BMSMODE  = BMS_MODE_E.BMS_FAULT;
      elseif t >= 8.6 && t < 10.6
      Expected_BMSMODE  = BMS_MODE_E.BMS_DISCHARGE;
      elseif t >= 10.6 && t < 20.6
      Expected_BMSMODE  = BMS_MODE_E.BMS_STANDBY;
      else
      Expected_BMSMODE  = BMS_MODE_E.BMS_SLEEP;
      end
      verify(AppOut_BMSMODE == Expected_BMSMODE );
    (default) -> SleepToDischgToFlt3.step_1
  state SleepToChgToFlt
    state step_1
      if t < 0.3
      Expected_BMSMODE  = BMS_MODE_E.BMS_SLEEP;
      elseif t >= 0.3 && t < 0.4
      Expected_BMSMODE  = BMS_MODE_E.BMS_STANDBY;
      elseif t >= 0.4 && t < 2.5
      Expected_BMSMODE  = BMS_MODE_E.BMS_CHARGE;
      elseif t >= 2.5 && t < 4.5
      Expected_BMSMODE  = BMS_MODE_E.BMS_FAULT;
      elseif t >= 4.5 && t < 6.5
      Expected_BMSMODE  = BMS_MODE_E.BMS_CHARGE;
      elseif t >= 6.5 && t < 16.5
      Expected_BMSMODE  = BMS_MODE_E.BMS_STANDBY;
      else
      Expected_BMSMODE  = BMS_MODE_E.BMS_SLEEP;
      end
      verify(AppOut_BMSMODE == Expected_BMSMODE );
    (default) -> SleepToChgToFlt.step_1
  state SleepToChgToFltToDischg
    state step_1
      if t < 0.3
      Expected_BMSMODE  = BMS_MODE_E.BMS_SLEEP;
      elseif t >= 0.3 && t < 0.4
      Expected_BMSMODE  = BMS_MODE_E.BMS_STANDBY;
      elseif t >= 0.4 && t < 2.5
      Expected_BMSMODE  = BMS_MODE_E.BMS_CHARGE;
      elseif t >= 2.5 && t < 3.5
      Expected_BMSMODE  = BMS_MODE_E.BMS_FAULT;
      elseif t >= 3.5 && t < 5.5
      Expected_BMSMODE  = BMS_MODE_E.BMS_DISCHARGE;
      elseif t >= 5.5 && t < 5.6
      Expected_BMSMODE  = BMS_MODE_E.BMS_STANDBY;
      elseif t >= 5.6 && t < 15.6
      Expected_BMSMODE  = BMS_MODE_E.BMS_FAULT;
      else
      Expected_BMSMODE  = BMS_MODE_E.BMS_SLEEP;
      end
      verify(AppOut_BMSMODE == Expected_BMSMODE );
    (default) -> SleepToChgToFltToDischg.step_1
  state SleepToChgToFltToDischg1
    state step_1
      if t < 0.3
      Expected_BMSMODE  = BMS_MODE_E.BMS_SLEEP;
      elseif t >= 0.3 && t < 0.4
      Expected_BMSMODE  = BMS_MODE_E.BMS_STANDBY;
      elseif t >= 0.4 && t < 2.5
      Expected_BMSMODE  = BMS_MODE_E.BMS_CHARGE;
      elseif t >= 2.5 && t < 3.5
      Expected_BMSMODE  = BMS_MODE_E.BMS_FAULT;
      elseif t >= 3.5 && t < 5.5
      Expected_BMSMODE  = BMS_MODE_E.BMS_DISCHARGE;
      elseif t >= 5.5 && t < 5.8
      Expected_BMSMODE  = BMS_MODE_E.BMS_STANDBY;
      elseif t >= 5.8 && t < 15.8
      Expected_BMSMODE  = BMS_MODE_E.BMS_FAULT;
      else
      Expected_BMSMODE  = BMS_MODE_E.BMS_SLEEP;
      end
      verify(AppOut_BMSMODE == Expected_BMSMODE );
    (default) -> SleepToChgToFltToDischg1.step_1
  state SleepToDischgToFltToChg
    state step_1
      if t < 0.3
      Expected_BMSMODE  = BMS_MODE_E.BMS_SLEEP;
      elseif t >= 0.3 && t < 0.4
      Expected_BMSMODE  = BMS_MODE_E.BMS_STANDBY;
      elseif t >= 0.4 && t < 2.5
      Expected_BMSMODE  = BMS_MODE_E.BMS_DISCHARGE;
      elseif t >= 2.5 && t < 3.5
      Expected_BMSMODE  = BMS_MODE_E.BMS_FAULT;
      elseif t >= 3.5 && t < 5.5
      Expected_BMSMODE  = BMS_MODE_E.BMS_CHARGE;
      elseif t >= 5.5 && t < 5.6
      Expected_BMSMODE  = BMS_MODE_E.BMS_STANDBY;
      elseif t >= 5.6 && t < 15.6
      Expected_BMSMODE  = BMS_MODE_E.BMS_FAULT;
      else
      Expected_BMSMODE  = BMS_MODE_E.BMS_SLEEP;
      end
      verify(AppOut_BMSMODE == Expected_BMSMODE );
    (default) -> SleepToDischgToFltToChg.step_1
  state SleepToDischgToFltToChg1
    state step_1
      if t < 0.3
      Expected_BMSMODE  = BMS_MODE_E.BMS_SLEEP;
      elseif t >= 0.3 && t < 0.4
      Expected_BMSMODE  = BMS_MODE_E.BMS_STANDBY;
      elseif t >= 0.4 && t < 2.5
      Expected_BMSMODE  = BMS_MODE_E.BMS_DISCHARGE;
      elseif t >= 2.5 && t < 3.5
      Expected_BMSMODE  = BMS_MODE_E.BMS_FAULT;
      elseif t >= 3.5 && t < 5.5
      Expected_BMSMODE  = BMS_MODE_E.BMS_CHARGE;
      elseif t >= 5.5 && t < 5.6
      Expected_BMSMODE  = BMS_MODE_E.BMS_STANDBY;
      elseif t >= 5.6 && t < 15.6
      Expected_BMSMODE  = BMS_MODE_E.BMS_FAULT;
      else
      Expected_BMSMODE  = BMS_MODE_E.BMS_SLEEP;
      end
      verify(AppOut_BMSMODE == Expected_BMSMODE );
    (default) -> SleepToDischgToFltToChg1.step_1
  state SleepToDischgToFltToChg2
    state step_1
      if t < 0.3
      Expected_BMSMODE  = BMS_MODE_E.BMS_SLEEP;
      elseif t >= 0.3 && t < 0.4
      Expected_BMSMODE  = BMS_MODE_E.BMS_STANDBY;
      elseif t >= 0.4 && t < 2.5
      Expected_BMSMODE  = BMS_MODE_E.BMS_DISCHARGE;
      elseif t >= 2.5 && t < 3.5
      Expected_BMSMODE  = BMS_MODE_E.BMS_FAULT;
      elseif t >= 3.5 && t < 5.5
      Expected_BMSMODE  = BMS_MODE_E.BMS_CHARGE;
      elseif t >= 5.5 && t < 5.6
      Expected_BMSMODE  = BMS_MODE_E.BMS_STANDBY;
      elseif t >= 5.6 && t < 15.6
      Expected_BMSMODE  = BMS_MODE_E.BMS_FAULT;
      else
      Expected_BMSMODE  = BMS_MODE_E.BMS_SLEEP;
      end
      verify(AppOut_BMSMODE == Expected_BMSMODE );
    (default) -> SleepToDischgToFltToChg2.step_1
  state ChargingSequence
    state step_1
      if t < 0.2
      Expected_BMSMODE  = BMS_MODE_E.BMS_SLEEP;
      elseif t >= 0.2 && t < 0.3
      Expected_BMSMODE  = BMS_MODE_E.BMS_STANDBY;
      elseif t >= 0.3 && t < 11.5
      Expected_BMSMODE  = BMS_MODE_E.BMS_CHARGE;
      elseif t >= 11.5 && t < 21.5
      Expected_BMSMODE  = BMS_MODE_E.BMS_STANDBY;
      else
      Expected_BMSMODE  = BMS_MODE_E.BMS_SLEEP;
      end
      if t < 0.3
      Expected_ChgModeReq = Charger_Mode_Req_E.Disabled;
      elseif t >= 0.3 && t < 1.4
      Expected_ChgModeReq = Charger_Mode_Req_E.Standby;
      elseif t >= 1.4 && t < 5.2
      Expected_ChgModeReq = Charger_Mode_Req_E.CC_Start;
      elseif t >= 5.2 && t < 8.2
      Expected_ChgModeReq = Charger_Mode_Req_E.CC_End;
      elseif t >= 8.2 && t < 11.5
      Expected_ChgModeReq = Charger_Mode_Req_E.CV;
      else
      Expected_ChgModeReq = Charger_Mode_Req_E.Disabled;
      end
      if t < 1.4
      Expected_ChargeVoltageLt = 0;
      elseif t >= 1.4 && t < 5.2
      Expected_ChargeVoltageLt = 85;
      elseif t >= 5.2 && t < 8.2
      Expected_ChargeVoltageLt = 0;
      elseif t >= 8.2 && t < 11.5
      Expected_ChargeVoltageLt = 85;
      else
      Expected_ChargeVoltageLt = 0;
      end
      if t < 1.4
      Expected_ChargeCurrentLt= 0;
      elseif t >= 1.4 && t < 5.2
      Expected_ChargeCurrentLt= 10;
      elseif t >= 5.2 && t < 8.2
      Expected_ChargeCurrentLt= 0;
      elseif t >= 8.2 && t < 11.5
      Expected_ChargeCurrentLt= 2.0;
      else
      Expected_ChargeCurrentLt= 0;
      end
      verify(AppOut_BMSMODE == Expected_BMSMODE );
      verify(AppOut_ChgModeReq== Expected_ChgModeReq);
      verify(AppOut_ChargeVoltageLt== Expected_ChargeVoltageLt);
      verify(AppOut_ChargeCurrentLt== Expected_ChargeCurrentLt);
    (default) -> ChargingSequence.step_1
  state ChargeSeq
    state step_1
      if t < 0.2
      Expected_BMSMODE  = BMS_MODE_E.BMS_SLEEP;
      elseif t >= 0.2 && t < 0.3
      Expected_BMSMODE  = BMS_MODE_E.BMS_STANDBY;
      elseif t >= 0.3 && t < 13.4
      Expected_BMSMODE  = BMS_MODE_E.BMS_CHARGE;
      elseif t >= 13.4 && t < 23.4
      Expected_BMSMODE  = BMS_MODE_E.BMS_STANDBY;
      else
      Expected_BMSMODE  = BMS_MODE_E.BMS_SLEEP;
      end
      if t < 0.3
      Expected_ChgModeReq = Charger_Mode_Req_E.Disabled;
      elseif t >= 0.3 && t < 1.4
      Expected_ChgModeReq = Charger_Mode_Req_E.Standby;
      elseif t >= 1.4 && t < 5.2
      Expected_ChgModeReq = Charger_Mode_Req_E.CC_Start;
      elseif t >= 5.2 && t < 8.2
      Expected_ChgModeReq = Charger_Mode_Req_E.CC_End;
      elseif t >= 8.2 && t < 13.3
      Expected_ChgModeReq = Charger_Mode_Req_E.CV;
      else
      Expected_ChgModeReq = Charger_Mode_Req_E.Charge_Complete;
      end
      if t < 1.4
      Expected_ChargeVoltageLt = 0;
      elseif t >= 1.4 && t < 5.2
      Expected_ChargeVoltageLt = 85;
      elseif t >= 5.2 && t < 8.2
      Expected_ChargeVoltageLt = 0;
      elseif t >= 8.2 && t < 13.3
      Expected_ChargeVoltageLt = 85;
      else
      Expected_ChargeVoltageLt = 0;
      end
      if t < 1.4
      Expected_ChargeCurrentLt= 0;
      elseif t >= 1.4 && t < 5.2
      Expected_ChargeCurrentLt= 10;
      elseif t >= 5.2 && t < 8.2
      Expected_ChargeCurrentLt= 0;
      elseif t >= 8.2 && t < 13.3
      Expected_ChargeCurrentLt= 2.0;
      else
      Expected_ChargeCurrentLt= 0;
      end
      verify(AppOut_BMSMODE == Expected_BMSMODE );
      verify(AppOut_ChgModeReq== Expected_ChgModeReq);
      verify(AppOut_ChargeVoltageLt== Expected_ChargeVoltageLt);
      verify(AppOut_ChargeCurrentLt== Expected_ChargeCurrentLt);
    (default) -> ChargeSeq.step_1
  state ChargeSeqG2Fault
    state step_1
      if t < 0.2
      Expected_BMSMODE  = BMS_MODE_E.BMS_SLEEP;
      elseif t >= 0.2 && t < 0.3
      Expected_BMSMODE  = BMS_MODE_E.BMS_STANDBY;
      elseif t >= 0.3 && t < 13.4
      Expected_BMSMODE  = BMS_MODE_E.BMS_CHARGE;
      elseif t >= 13.4 && t < 23.4
      Expected_BMSMODE  = BMS_MODE_E.BMS_STANDBY;
      else
      Expected_BMSMODE  = BMS_MODE_E.BMS_SLEEP;
      end
      if t < 0.3
      Expected_ChgModeReq = Charger_Mode_Req_E.Disabled;
      elseif t >= 0.3 && t < 1.4
      Expected_ChgModeReq = Charger_Mode_Req_E.Standby;
      elseif t >= 1.4 && t < 5.2
      Expected_ChgModeReq = Charger_Mode_Req_E.CC_Start;
      elseif t >= 5.2 && t < 8.2
      Expected_ChgModeReq = Charger_Mode_Req_E.CC_End;
      elseif t >= 8.2 && t < 13.3
      Expected_ChgModeReq = Charger_Mode_Req_E.CV;
      else
      Expected_ChgModeReq = Charger_Mode_Req_E.Charge_Complete;
      end
      if t < 1.4
      Expected_ChargeVoltageLt = 0;
      elseif t >= 1.4 && t < 5.2
      Expected_ChargeVoltageLt = 85;
      elseif t >= 5.2 && t < 8.2
      Expected_ChargeVoltageLt = 0;
      elseif t >= 8.2 && t < 13.3
      Expected_ChargeVoltageLt = 85;
      else
      Expected_ChargeVoltageLt = 0;
      end
      if t < 1.4
      Expected_ChargeCurrentLt= 0;
      elseif t >= 1.4 && t < 5.2
      Expected_ChargeCurrentLt= 5;
      elseif t >= 5.2 && t < 8.2
      Expected_ChargeCurrentLt= 0;
      elseif t >= 8.2 && t < 13.3
      Expected_ChargeCurrentLt= 2.0;
      else
      Expected_ChargeCurrentLt= 0;
      end
      verify(AppOut_BMSMODE == Expected_BMSMODE);
      verify(AppOut_ChgModeReq== Expected_ChgModeReq);
      verify(AppOut_ChargeVoltageLt== Expected_ChargeVoltageLt);
      verify(AppOut_ChargeCurrentLt== Expected_ChargeCurrentLt);
    (default) -> ChargeSeqG2Fault.step_1
  state ChargeSeq1
    state step_1
      if t < 0.2
      Expected_BMSMODE  = BMS_MODE_E.BMS_SLEEP;
      elseif t >= 0.2 && t < 0.3
      Expected_BMSMODE  = BMS_MODE_E.BMS_STANDBY;
      elseif t >= 0.3 && t < 13.4
      Expected_BMSMODE  = BMS_MODE_E.BMS_CHARGE;
      else
      Expected_BMSMODE  = BMS_MODE_E.BMS_STANDBY;
      end
      if t < 0.3
      Expected_ChgModeReq = Charger_Mode_Req_E.Disabled;
      elseif t >= 0.3 && t < 1.4
      Expected_ChgModeReq = Charger_Mode_Req_E.Standby;
      elseif t >= 1.4 && t < 5.2
      Expected_ChgModeReq = Charger_Mode_Req_E.CC_Start;
      elseif t >= 5.2 && t < 8.2
      Expected_ChgModeReq = Charger_Mode_Req_E.CC_End;
      elseif t >= 8.2 && t < 13.3
      Expected_ChgModeReq = Charger_Mode_Req_E.CV;
      else
      Expected_ChgModeReq = Charger_Mode_Req_E.Charge_Complete;
      end
      if t < 1.4
      Expected_ChargeVoltageLt = 0;
      elseif t >= 1.4 && t < 5.2
      Expected_ChargeVoltageLt = 85;
      elseif t >= 5.2 && t < 8.2
      Expected_ChargeVoltageLt = 0;
      elseif t >= 8.2 && t < 13.3
      Expected_ChargeVoltageLt = 85;
      else
      Expected_ChargeVoltageLt = 0;
      end
      if t < 1.4
      Expected_ChargeCurrentLt= 0;
      elseif t >= 1.4 && t < 5.2
      Expected_ChargeCurrentLt= 10;
      elseif t >= 5.2 && t < 8.2
      Expected_ChargeCurrentLt= 0;
      elseif t >= 8.2 && t < 13.3
      Expected_ChargeCurrentLt= 2.0;
      else
      Expected_ChargeCurrentLt= 0;
      end
      verify(AppOut_BMSMODE == Expected_BMSMODE );
      verify(AppOut_ChgModeReq== Expected_ChgModeReq);
      verify(AppOut_ChargeVoltageLt== Expected_ChargeVoltageLt);
      verify(AppOut_ChargeCurrentLt== Expected_ChargeCurrentLt);
    (default) -> ChargeSeq1.step_1
  (default) -> ChargeWhenIgOn [order 1] : [Active_Scenario_Index == 1]
  (default) -> DischgWhenIgOn [order 2] : [Active_Scenario_Index == 2]
  (default) -> ChargeWhenIgOff [order 3] : [Active_Scenario_Index == 3]
  (default) -> ChgToDischgIgOn [order 4] : [Active_Scenario_Index == 4]
  (default) -> SleepToStandby [order 5] : [Active_Scenario_Index == 5]
  (default) -> DischgToStandby [order 6] : [Active_Scenario_Index == 6]
  (default) -> StandbyToDischgIgOn [order 7] : [Active_Scenario_Index == 7]
  (default) -> IgOffToOnInCharge [order 8] : [Active_Scenario_Index == 8]
  (default) -> IgOnToOffInCharge [order 9] : [Active_Scenario_Index == 9]
  (default) -> VehPoweredOff [order 10] : [Active_Scenario_Index == 10]
  (default) -> G4T1DischgFlt [order 11] : [Active_Scenario_Index == 11]
  (default) -> G4T2DischgFlt [order 12] : [Active_Scenario_Index == 12]
  (default) -> G4CommonFlt [order 13] : [Active_Scenario_Index == 13]
  (default) -> G4ChargeFlt [order 14] : [Active_Scenario_Index == 14]
  (default) -> DischgToChgIgOn [order 15] : [Active_Scenario_Index == 15]
  (default) -> FaultToSleep [order 16] : [Active_Scenario_Index == 16]
  (default) -> ChgToStandbyIgOn [order 17] : [Active_Scenario_Index == 17]
  (default) -> ChgToStandbyIgOff [order 18] : [Active_Scenario_Index == 18]
  (default) -> StandbyToChargeIgOn [order 19] : [Active_Scenario_Index == 19]
  (default) -> StandbyToChargeIgOff [order 20] : [Active_Scenario_Index == 20]
  (default) -> ChgToFltIgOff [order 21] : [Active_Scenario_Index == 21]
  (default) -> FltToChgIgOff [order 22] : [Active_Scenario_Index == 22]
  (default) -> FltToChgIgOn [order 23] : [Active_Scenario_Index == 23]
  (default) -> PrechgVoltFltWhenIgOn [order 24] : [Active_Scenario_Index == 24]
  (default) -> PrechgVoltFltWhenIgOff [order 25] : [Active_Scenario_Index == 25]
  (default) -> ChargeSequenceIgOff [order 26] : [Active_Scenario_Index == 26]
  (default) -> ChargeSequenceIgOn [order 27] : [Active_Scenario_Index == 27]
  (default) -> DischgToChargeAndIgOnToOff [order 28] : [Active_Scenario_Index == 28]
  (default) -> G4T2DischargeToSleep [order 29] : [Active_Scenario_Index == 29]
  (default) -> G4Typ2DischgToSleep [order 30] : [Active_Scenario_Index == 30]
  (default) -> G4T1DischargeToSleep [order 31] : [Active_Scenario_Index == 31]
  (default) -> G4Typ1DischgToSleep [order 32] : [Active_Scenario_Index == 32]
  (default) -> G4CommonToSleep [order 33] : [Active_Scenario_Index == 33]
  (default) -> G4CommToSleep [order 34] : [Active_Scenario_Index == 34]
  (default) -> G4ChargeToSleep [order 35] : [Active_Scenario_Index == 35]
  (default) -> G4ChgToSleep [order 36] : [Active_Scenario_Index == 36]
  (default) -> ChgToDischgToSleep [order 37] : [Active_Scenario_Index == 37]
  (default) -> G4CommToChg [order 38] : [Active_Scenario_Index == 38]
  (default) -> G4ChgFltToDischg [order 39] : [Active_Scenario_Index == 39]
  (default) -> G4T1DischgToG4T2Dischg [order 40] : [Active_Scenario_Index == 40]
  (default) -> SleepToCharge [order 41] : [Active_Scenario_Index == 41]
  (default) -> SleepToDischarge [order 42] : [Active_Scenario_Index == 42]
  (default) -> SleepToChargeToSleep [order 43] : [Active_Scenario_Index == 43]
  (default) -> SleepToChg [order 44] : [Active_Scenario_Index == 44]
  (default) -> SleepToChrg [order 45] : [Active_Scenario_Index == 45]
  (default) -> SleepToStbToG3CommFlt [order 46] : [Active_Scenario_Index == 46]
  (default) -> SleepToStbToG4CommFlt [order 47] : [Active_Scenario_Index == 47]
  (default) -> SleepToStbToG4CommFlt1 [order 48] : [Active_Scenario_Index == 48]
  (default) -> SleepToDischgToFlt [order 49] : [Active_Scenario_Index == 49]
  (default) -> SleepToDischgToFlt1 [order 50] : [Active_Scenario_Index == 50]
  (default) -> SleepToDischgToFlt2 [order 51] : [Active_Scenario_Index == 51]
  (default) -> SleepToDischgToFlt3 [order 52] : [Active_Scenario_Index == 52]
  (default) -> SleepToChgToFlt [order 53] : [Active_Scenario_Index == 53]
  (default) -> SleepToChgToFltToDischg [order 54] : [Active_Scenario_Index == 54]
  (default) -> SleepToChgToFltToDischg1 [order 55] : [Active_Scenario_Index == 55]
  (default) -> SleepToDischgToFltToChg [order 56] : [Active_Scenario_Index == 56]
  (default) -> SleepToDischgToFltToChg1 [order 57] : [Active_Scenario_Index == 57]
  (default) -> SleepToDischgToFltToChg2 [order 58] : [Active_Scenario_Index == 58]
  (default) -> ChargingSequence [order 59] : [Active_Scenario_Index == 59]
  (default) -> ChargeSeq [order 60] : [Active_Scenario_Index == 60]
  (default) -> ChargeSeqG2Fault [order 61] : [Active_Scenario_Index == 61]
  (default) -> ChargeSeq1 [order 62] : {assert(Active_Scenario_Index == 62,'The value of Scenario Parameter ''Active_Scenario_Index'' is not valid. Use the index of the scenario to specify it.')}
  data: AppOut_BMSMODE input; AppOut_PrechgMosfetCmd input; AppOut_HVMosfetCmd input; AppOut_DCDCMosfetCmd input; AppOut_PrechgMosfet input; AppOut_HVMosfet input; AppOut_DCDCMosfet input; AppOut_ASC_Prep_Flag input; AppOut_Chrgr_Prep_Flag input; AppOut_PrechgVoltFlt input; AppOut_ChgModeReq input; AppOut_ChargeVoltageLt input; AppOut_ChargeCurrentLt input; AppOut_DisplaySoC input; AppOut_BatteryCapacity input; AppOut_LowSoCWarn15 input; AppOut_LowSoC input; AppOut_LowSoCWarn input; AppOut_BattPackSOC input; AppOut_LifeCycle input; AppOut_SOH input; AppOut_CurrentCapacity input; AppOut_SOCcc input; AppOut_SOCocvavg input; AppOut_SOCocvInit input; AppOut_SOCAvgInitial input; AppOut_AvailableEnergy input; AppOut_ChargeCapacity input; AppOut_DischgCurrLimit input; AppOut_Timer30 input; AppOut_BMS_NM_Msg input; AppOut_RegenOverCurrentFlg input; AppOut_RegenCurrent input size=[1*1]; AppOut_DerateFlg input; Expected_BMSMODE output Enum: BMS_MODE_E; Expected_PrechgMosfet output Enum: BMS_PMosfet_STS_E; Expected_HVMosfet output Enum: BMS_HVMosfet_STS_E; Expected_DCDCMosfet output Enum: BMS_DCDCMosfet_STS_E; Expected_ASC_Prep_Flag output boolean; Expected_Chrgr_Prep_Flag output boolean; Expected_PrechgVoltFlt output boolean; Active_Scenario_Index parameter; AppOut_BattTempDerating input; AppOut_BattSoCDerating input; Expected_ChgModeReq output; Expected_ChargeVoltageLt output; Expected_ChargeCurrentLt output
